simulink model "rfsoc4x2_ospfb_128"  (R2021a)
settings: Solver=VariableStepAuto  StartTime=0.0  StopTime=2048  RelTol=1e-3
undefined symbols (not defined in the file): pfb_coeff_gen_calc
libraries: xbsIndex_r4 x37092, casper_library_delays x737, casper_library_misc x68, xps_library x1
(part 15 of 339)

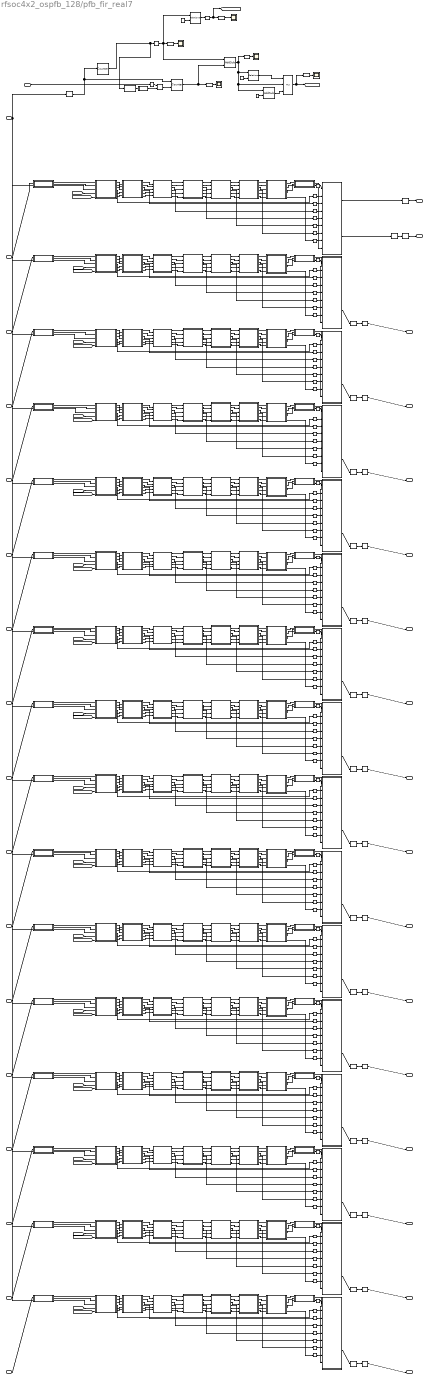
== system rfsoc4x2_ospfb_128/pfb_fir_real7 ==
  note: data 9 first out
  sync : Inport
  pol1_in1 : Inport  Port=2
  pol1_in2 : Inport  Port=3
  pol1_in3 : Inport  Port=4
  pol1_in4 : Inport  Port=5
  pol1_in5 : Inport  Port=6
  pol1_in6 : Inport  Port=7
  pol1_in7 : Inport  Port=8
  pol1_in8 : Inport  Port=9
  pol1_in9 : Inport  Port=10
  pol1_in10 : Inport  Port=11
  pol1_in11 : Inport  Port=12
  pol1_in12 : Inport  Port=13
  pol1_in13 : Inport  Port=14
  pol1_in14 : Inport  Port=15
  pol1_in15 : Inport  Port=16
  pol1_in16 : Inport  Port=17
  en_ctrl : Inport  Port=18
  AddSub11 : xbsIndex_r4/AddSub  mode=Addition  use_carryin=off  use_carryout=off  en=off  latency=0  precision=User Defined  arith_type=Unsigned  n_bits=(log2((2^8 / 2^4)))+1  bin_pt=0  quantization=Truncate  overflow=Wrap  use_behavioral_HDL=off  hw_selection=Fabric  pipelined=off  dbl_ovrd=off  block_type=addsub
  AddSub12 : xbsIndex_r4/AddSub  mode=Subtraction  use_carryin=off  use_carryout=off  en=off  latency=0  precision=User Defined  arith_type=Unsigned  n_bits=log2((2^8 / 2^4))  bin_pt=0  quantization=Truncate  overflow=Wrap  use_behavioral_HDL=off  hw_selection=Fabric  pipelined=off  dbl_ovrd=off  block_type=addsub
  Constant61 : xbsIndex_r4/Constant  const=(2^8 / 2^4) - 1  gui_display_data_type=Fixed-point  arith_type=Unsigned  n_bits=log2((2^8 / 2^4))  bin_pt=0  preci_type=Single  exp_width=8  frac_width=24  explicit_period=off  period=1  equ=P=C  opselect=C  inp2=PCIN>>17  opr=+  inp1=P  carry=CIN  dbl_ovrd=off  block_type=constant
  Constant62 : xbsIndex_r4/Constant  const=(2^8 / 2^4)  gui_display_data_type=Fixed-point  arith_type=Unsigned  n_bits=log2((2^8 / 2^4)) + 1  bin_pt=0  preci_type=Single  exp_width=8  frac_width=24  explicit_period=off  period=1  equ=P=C  opselect=C  inp2=PCIN>>17  opr=+  inp1=P  carry=CIN  dbl_ovrd=off  block_type=constant
  Constant63 : xbsIndex_r4/Constant  const=11  gui_display_data_type=Fixed-point  arith_type=Unsigned  n_bits=4  bin_pt=0  preci_type=Single  exp_width=8  frac_width=24  explicit_period=off  period=1  equ=P=C  opselect=C  inp2=PCIN>>17  opr=+  inp1=P  carry=CIN  dbl_ovrd=off  block_type=constant
  Counter36 : xbsIndex_r4/Counter  cnt_type=Free Running  cnt_to=1023  operation=Down  start_count=0  cnt_by_val=(2^8 / 2^4)/4  arith_type=Unsigned  n_bits=log2((2^8 / 2^4))  bin_pt=0  load_pin=off  rst=on  en=on  explicit_period=on  period=1  use_behavioral_HDL=off  implementation=Fabric  dbl_ovrd=off  block_type=counter
  Counter38 : xbsIndex_r4/Counter  cnt_type=Free Running  cnt_to=1023  operation=Up  start_count=0  cnt_by_val=1  arith_type=Unsigned  n_bits=log2((2^8 / 2^4))  bin_pt=0  load_pin=off  rst=on  en=off  explicit_period=on  period=1  use_behavioral_HDL=off  implementation=Fabric  dbl_ovrd=off  block_type=counter
  Delay26 : xbsIndex_r4/Delay  rst=off  infoeditControl=Selection of Reset will increase slice count due to use of real FFs and instead of SRLs  en=off  latency=1  reg_retiming=off  dbl_ovrd=off  block_type=delay
  Delay27 : xbsIndex_r4/Delay  rst=off  infoeditControl=Selection of Reset will increase slice count due to use of real FFs and instead of SRLs  en=off  latency=4  reg_retiming=off  dbl_ovrd=off  block_type=delay
  Gateway Out{250..253,255} (5 alike) : xbsIndex_r4/Gateway Out  inherit_from_input=off  hdl_port=on  rows=1  columns=1  UseAsDAC=off  DACChannel='1'  interface=None  automatic_assignment=on  address_offset=hex2dec('00')  intf_name=''  intf_description=''  timing_constraint=None  locs_specified=off  LOCs={}  io_standard={}  block_type=gatewayout
  Inverter : xbsIndex_r4/Inverter  en=off  latency=0  dbl_ovrd=off  block_type=inv
  Logical11 : xbsIndex_r4/Logical  logical_function=AND  inputs=2  en=off  latency=0  precision=Full  arith_type=Unsigned  n_bits=16  bin_pt=0  align_bp=on  dbl_ovrd=off  block_type=logical
  Mux3 : xbsIndex_r4/Mux  inputs=2  en=off  latency=0  precision=User Defined  arith_type=Unsigned  n_bits=log2((2^8 / 2^4))  bin_pt=0  quantization=Truncate  overflow=Wrap  dbl_ovrd=off  block_type=mux
  Relational11 : xbsIndex_r4/Relational  mode=a>b  op_type=Bool  en=off  latency=0  dbl_ovrd=off  block_type=relational
  Relational12 : xbsIndex_r4/Relational  mode=a>b  op_type=Bool  en=off  latency=0  dbl_ovrd=off  block_type=relational
  Slice20 : xbsIndex_r4/Slice  nbits=1  boolean_output=on  mode=Upper Bit Location + Width  bit1=0  base1=MSB of Input  bit0=0  base0=LSB of Input  dbl_ovrd=off  block_type=slice
  adder_1_1 : Subsystem  AncestorBlock=casper_library_misc/adder_tree  mask(adder_tree){n_inputs=8, csp_latency=1, adder_imp=Fabric, first_stage_hdl=on, floating_point=off, dvalid_en=off, float_type=single, frac_width=0, exp_width=0}
      mask prompts: n_inputs "Number of Inputs"; csp_latency "Add Latency"; adder_imp "Adder implementation"; first_stage_hdl "Use behavioural HDL for first stage of adders"; floating_point "floating point"; float_type "float type"; frac_width "fraction length"; exp_width "exponent length"
      mask help:
      | Sums all inputs using a tree of adds and delays.
      |
      | Number of inputs: The number of inputs to the block to be summed
      | Add latency: The number of clock cycles to perform one addition (affects timing)..
      | Adder implementation: choice of fabric or DSP48E core, or behavioral HDL
      | Use behavioural HDL for first stage of adders: Causes the first stage of adders to be absorbed into DSP blocks if multipliers precede them (Virtex 5). Overrides Adder implementation
      mask init: same as rfsoc4x2_ospfb_128/pfb_fir_real10/adder_1_1
      settings: AttributesFormatString=latency 3
      mask Help: eval('xlWeb(''http://casper.berkeley.edu/wiki/Adder_tree'')')
      mask TypeOptions adder_imp: Behavioral | Fabric | DSP48
      mask Callback floating_point:
      | onoff = get_param(gcb, 'floating_point');
      | if strcmp(onoff,'on')
      |     enable_fixpt = 'off';
      |     set_param_state(gcb, 'float_type', 'on')
      | 
      |     f_type = get_param(gcb, 'float_type');
      |     if strcmp(f_type,'custom')
      |         set_param_state(gcb, 'exp_width', 'on')
      |         set_param_state(gcb, 'frac_width', 'on')
      |     else
      |         set_param_state(gcb, 'exp_width', 'off')
      |         set_param_state(gcb, 'frac_width', 'off')
      |     end
      | 
      | 
      | else
      |     enable_fixpt = 'on';
      |     set_param_state(gcb, 'float_type', 'off')
      |     set_param_state(gcb, 'exp_width', 'off')
      |     set_param_state(gcb, 'frac_width', 'off')
      | end
      mask TypeOptions float_type: single | custom
      mask Callback float_type:
      | f_type = get_param(gcb, 'float_type');
      | if strcmp(f_type,'custom')
      |     set_param_state(gcb, 'exp_width', 'on')
      |     set_param_state(gcb, 'frac_width', 'on')
      | else
      |     set_param_state(gcb, 'exp_width', 'off')
      |     set_param_state(gcb, 'frac_width', 'off')
      | end
  adder_1_10 : Subsystem  AncestorBlock=casper_library_misc/adder_tree  mask(adder_tree){n_inputs=8, csp_latency=1, adder_imp=Fabric, first_stage_hdl=on, floating_point=off, dvalid_en=off, float_type=single, frac_width=0, exp_width=0}
      mask prompts: n_inputs "Number of Inputs"; csp_latency "Add Latency"; adder_imp "Adder implementation"; first_stage_hdl "Use behavioural HDL for first stage of adders"; floating_point "floating point"; float_type "float type"; frac_width "fraction length"; exp_width "exponent length"
      mask help:
      | Sums all inputs using a tree of adds and delays.
      |
      | Number of inputs: The number of inputs to the block to be summed
      | Add latency: The number of clock cycles to perform one addition (affects timing)..
      | Adder implementation: choice of fabric or DSP48E core, or behavioral HDL
      | Use behavioural HDL for first stage of adders: Causes the first stage of adders to be absorbed into DSP blocks if multipliers precede them (Virtex 5). Overrides Adder implementation
      mask init: same as rfsoc4x2_ospfb_128/pfb_fir_real10/adder_1_1
      settings: AttributesFormatString=latency 3
      mask Help: eval('xlWeb(''http://casper.berkeley.edu/wiki/Adder_tree'')')
      mask TypeOptions adder_imp: Behavioral | Fabric | DSP48
      mask Callback floating_point:
      | onoff = get_param(gcb, 'floating_point');
      | if strcmp(onoff,'on')
      |     enable_fixpt = 'off';
      |     set_param_state(gcb, 'float_type', 'on')
      | 
      |     f_type = get_param(gcb, 'float_type');
      |     if strcmp(f_type,'custom')
      |         set_param_state(gcb, 'exp_width', 'on')
      |         set_param_state(gcb, 'frac_width', 'on')
      |     else
      |         set_param_state(gcb, 'exp_width', 'off')
      |         set_param_state(gcb, 'frac_width', 'off')
      |     end
      | 
      | 
      | else
      |     enable_fixpt = 'on';
      |     set_param_state(gcb, 'float_type', 'off')
      |     set_param_state(gcb, 'exp_width', 'off')
      |     set_param_state(gcb, 'frac_width', 'off')
      | end
      mask TypeOptions float_type: single | custom
      mask Callback float_type:
      | f_type = get_param(gcb, 'float_type');
      | if strcmp(f_type,'custom')
      |     set_param_state(gcb, 'exp_width', 'on')
      |     set_param_state(gcb, 'frac_width', 'on')
      | else
      |     set_param_state(gcb, 'exp_width', 'off')
      |     set_param_state(gcb, 'frac_width', 'off')
      | end
  adder_1_11 : Subsystem  AncestorBlock=casper_library_misc/adder_tree  mask(adder_tree){n_inputs=8, csp_latency=1, adder_imp=Fabric, first_stage_hdl=on, floating_point=off, dvalid_en=off, float_type=single, frac_width=0, exp_width=0}
      mask prompts: n_inputs "Number of Inputs"; csp_latency "Add Latency"; adder_imp "Adder implementation"; first_stage_hdl "Use behavioural HDL for first stage of adders"; floating_point "floating point"; float_type "float type"; frac_width "fraction length"; exp_width "exponent length"
      mask help:
      | Sums all inputs using a tree of adds and delays.
      |
      | Number of inputs: The number of inputs to the block to be summed
      | Add latency: The number of clock cycles to perform one addition (affects timing)..
      | Adder implementation: choice of fabric or DSP48E core, or behavioral HDL
      | Use behavioural HDL for first stage of adders: Causes the first stage of adders to be absorbed into DSP blocks if multipliers precede them (Virtex 5). Overrides Adder implementation
      mask init: same as rfsoc4x2_ospfb_128/pfb_fir_real10/adder_1_1
      settings: AttributesFormatString=latency 3
      mask Help: eval('xlWeb(''http://casper.berkeley.edu/wiki/Adder_tree'')')
      mask TypeOptions adder_imp: Behavioral | Fabric | DSP48
      mask Callback floating_point:
      | onoff = get_param(gcb, 'floating_point');
      | if strcmp(onoff,'on')
      |     enable_fixpt = 'off';
      |     set_param_state(gcb, 'float_type', 'on')
      | 
      |     f_type = get_param(gcb, 'float_type');
      |     if strcmp(f_type,'custom')
      |         set_param_state(gcb, 'exp_width', 'on')
      |         set_param_state(gcb, 'frac_width', 'on')
      |     else
      |         set_param_state(gcb, 'exp_width', 'off')
      |         set_param_state(gcb, 'frac_width', 'off')
      |     end
      | 
      | 
      | else
      |     enable_fixpt = 'on';
      |     set_param_state(gcb, 'float_type', 'off')
      |     set_param_state(gcb, 'exp_width', 'off')
      |     set_param_state(gcb, 'frac_width', 'off')
      | end
      mask TypeOptions float_type: single | custom
      mask Callback float_type:
      | f_type = get_param(gcb, 'float_type');
      | if strcmp(f_type,'custom')
      |     set_param_state(gcb, 'exp_width', 'on')
      |     set_param_state(gcb, 'frac_width', 'on')
      | else
      |     set_param_state(gcb, 'exp_width', 'off')
      |     set_param_state(gcb, 'frac_width', 'off')
      | end
  adder_1_12 : Subsystem  AncestorBlock=casper_library_misc/adder_tree  mask(adder_tree){n_inputs=8, csp_latency=1, adder_imp=Fabric, first_stage_hdl=on, floating_point=off, dvalid_en=off, float_type=single, frac_width=0, exp_width=0}
      mask prompts: n_inputs "Number of Inputs"; csp_latency "Add Latency"; adder_imp "Adder implementation"; first_stage_hdl "Use behavioural HDL for first stage of adders"; floating_point "floating point"; float_type "float type"; frac_width "fraction length"; exp_width "exponent length"
      mask help:
      | Sums all inputs using a tree of adds and delays.
      |
      | Number of inputs: The number of inputs to the block to be summed
      | Add latency: The number of clock cycles to perform one addition (affects timing)..
      | Adder implementation: choice of fabric or DSP48E core, or behavioral HDL
      | Use behavioural HDL for first stage of adders: Causes the first stage of adders to be absorbed into DSP blocks if multipliers precede them (Virtex 5). Overrides Adder implementation
      mask init: same as rfsoc4x2_ospfb_128/pfb_fir_real10/adder_1_1
      settings: AttributesFormatString=latency 3
      mask Help: eval('xlWeb(''http://casper.berkeley.edu/wiki/Adder_tree'')')
      mask TypeOptions adder_imp: Behavioral | Fabric | DSP48
      mask Callback floating_point:
      | onoff = get_param(gcb, 'floating_point');
      | if strcmp(onoff,'on')
      |     enable_fixpt = 'off';
      |     set_param_state(gcb, 'float_type', 'on')
      | 
      |     f_type = get_param(gcb, 'float_type');
      |     if strcmp(f_type,'custom')
      |         set_param_state(gcb, 'exp_width', 'on')
      |         set_param_state(gcb, 'frac_width', 'on')
      |     else
      |         set_param_state(gcb, 'exp_width', 'off')
      |         set_param_state(gcb, 'frac_width', 'off')
      |     end
      | 
      | 
      | else
      |     enable_fixpt = 'on';
      |     set_param_state(gcb, 'float_type', 'off')
      |     set_param_state(gcb, 'exp_width', 'off')
      |     set_param_state(gcb, 'frac_width', 'off')
      | end
      mask TypeOptions float_type: single | custom
      mask Callback float_type:
      | f_type = get_param(gcb, 'float_type');
      | if strcmp(f_type,'custom')
      |     set_param_state(gcb, 'exp_width', 'on')
      |     set_param_state(gcb, 'frac_width', 'on')
      | else
      |     set_param_state(gcb, 'exp_width', 'off')
      |     set_param_state(gcb, 'frac_width', 'off')
      | end
  adder_1_13 : Subsystem  AncestorBlock=casper_library_misc/adder_tree  mask(adder_tree){n_inputs=8, csp_latency=1, adder_imp=Fabric, first_stage_hdl=on, floating_point=off, dvalid_en=off, float_type=single, frac_width=0, exp_width=0}
      mask prompts: n_inputs "Number of Inputs"; csp_latency "Add Latency"; adder_imp "Adder implementation"; first_stage_hdl "Use behavioural HDL for first stage of adders"; floating_point "floating point"; float_type "float type"; frac_width "fraction length"; exp_width "exponent length"
      mask help:
      | Sums all inputs using a tree of adds and delays.
      |
      | Number of inputs: The number of inputs to the block to be summed
      | Add latency: The number of clock cycles to perform one addition (affects timing)..
      | Adder implementation: choice of fabric or DSP48E core, or behavioral HDL
      | Use behavioural HDL for first stage of adders: Causes the first stage of adders to be absorbed into DSP blocks if multipliers precede them (Virtex 5). Overrides Adder implementation
      mask init: same as rfsoc4x2_ospfb_128/pfb_fir_real10/adder_1_1
      settings: AttributesFormatString=latency 3
      mask Help: eval('xlWeb(''http://casper.berkeley.edu/wiki/Adder_tree'')')
      mask TypeOptions adder_imp: Behavioral | Fabric | DSP48
      mask Callback floating_point:
      | onoff = get_param(gcb, 'floating_point');
      | if strcmp(onoff,'on')
      |     enable_fixpt = 'off';
      |     set_param_state(gcb, 'float_type', 'on')
      | 
      |     f_type = get_param(gcb, 'float_type');
      |     if strcmp(f_type,'custom')
      |         set_param_state(gcb, 'exp_width', 'on')
      |         set_param_state(gcb, 'frac_width', 'on')
      |     else
      |         set_param_state(gcb, 'exp_width', 'off')
      |         set_param_state(gcb, 'frac_width', 'off')
      |     end
      | 
      | 
      | else
      |     enable_fixpt = 'on';
      |     set_param_state(gcb, 'float_type', 'off')
      |     set_param_state(gcb, 'exp_width', 'off')
      |     set_param_state(gcb, 'frac_width', 'off')
      | end
      mask TypeOptions float_type: single | custom
      mask Callback float_type:
      | f_type = get_param(gcb, 'float_type');
      | if strcmp(f_type,'custom')
      |     set_param_state(gcb, 'exp_width', 'on')
      |     set_param_state(gcb, 'frac_width', 'on')
      | else
      |     set_param_state(gcb, 'exp_width', 'off')
      |     set_param_state(gcb, 'frac_width', 'off')
      | end
  adder_1_14 : Subsystem  AncestorBlock=casper_library_misc/adder_tree  mask(adder_tree){n_inputs=8, csp_latency=1, adder_imp=Fabric, first_stage_hdl=on, floating_point=off, dvalid_en=off, float_type=single, frac_width=0, exp_width=0}
      mask prompts: n_inputs "Number of Inputs"; csp_latency "Add Latency"; adder_imp "Adder implementation"; first_stage_hdl "Use behavioural HDL for first stage of adders"; floating_point "floating point"; float_type "float type"; frac_width "fraction length"; exp_width "exponent length"
      mask help:
      | Sums all inputs using a tree of adds and delays.
      |
      | Number of inputs: The number of inputs to the block to be summed
      | Add latency: The number of clock cycles to perform one addition (affects timing)..
      | Adder implementation: choice of fabric or DSP48E core, or behavioral HDL
      | Use behavioural HDL for first stage of adders: Causes the first stage of adders to be absorbed into DSP blocks if multipliers precede them (Virtex 5). Overrides Adder implementation
      mask init: same as rfsoc4x2_ospfb_128/pfb_fir_real10/adder_1_1
      settings: AttributesFormatString=latency 3
      mask Help: eval('xlWeb(''http://casper.berkeley.edu/wiki/Adder_tree'')')
      mask TypeOptions adder_imp: Behavioral | Fabric | DSP48
      mask Callback floating_point:
      | onoff = get_param(gcb, 'floating_point');
      | if strcmp(onoff,'on')
      |     enable_fixpt = 'off';
      |     set_param_state(gcb, 'float_type', 'on')
      | 
      |     f_type = get_param(gcb, 'float_type');
      |     if strcmp(f_type,'custom')
      |         set_param_state(gcb, 'exp_width', 'on')
      |         set_param_state(gcb, 'frac_width', 'on')
      |     else
      |         set_param_state(gcb, 'exp_width', 'off')
      |         set_param_state(gcb, 'frac_width', 'off')
      |     end
      | 
      | 
      | else
      |     enable_fixpt = 'on';
      |     set_param_state(gcb, 'float_type', 'off')
      |     set_param_state(gcb, 'exp_width', 'off')
      |     set_param_state(gcb, 'frac_width', 'off')
      | end
      mask TypeOptions float_type: single | custom
      mask Callback float_type:
      | f_type = get_param(gcb, 'float_type');
      | if strcmp(f_type,'custom')
      |     set_param_state(gcb, 'exp_width', 'on')
      |     set_param_state(gcb, 'frac_width', 'on')
      | else
      |     set_param_state(gcb, 'exp_width', 'off')
      |     set_param_state(gcb, 'frac_width', 'off')
      | end
  adder_1_15 : Subsystem  AncestorBlock=casper_library_misc/adder_tree  mask(adder_tree){n_inputs=8, csp_latency=1, adder_imp=Fabric, first_stage_hdl=on, floating_point=off, dvalid_en=off, float_type=single, frac_width=0, exp_width=0}
      mask prompts: n_inputs "Number of Inputs"; csp_latency "Add Latency"; adder_imp "Adder implementation"; first_stage_hdl "Use behavioural HDL for first stage of adders"; floating_point "floating point"; float_type "float type"; frac_width "fraction length"; exp_width "exponent length"
      mask help:
      | Sums all inputs using a tree of adds and delays.
      |
      | Number of inputs: The number of inputs to the block to be summed
      | Add latency: The number of clock cycles to perform one addition (affects timing)..
      | Adder implementation: choice of fabric or DSP48E core, or behavioral HDL
      | Use behavioural HDL for first stage of adders: Causes the first stage of adders to be absorbed into DSP blocks if multipliers precede them (Virtex 5). Overrides Adder implementation
      mask init: same as rfsoc4x2_ospfb_128/pfb_fir_real10/adder_1_1
      settings: AttributesFormatString=latency 3
      mask Help: eval('xlWeb(''http://casper.berkeley.edu/wiki/Adder_tree'')')
      mask TypeOptions adder_imp: Behavioral | Fabric | DSP48
      mask Callback floating_point:
      | onoff = get_param(gcb, 'floating_point');
      | if strcmp(onoff,'on')
      |     enable_fixpt = 'off';
      |     set_param_state(gcb, 'float_type', 'on')
      | 
      |     f_type = get_param(gcb, 'float_type');
      |     if strcmp(f_type,'custom')
      |         set_param_state(gcb, 'exp_width', 'on')
      |         set_param_state(gcb, 'frac_width', 'on')
      |     else
      |         set_param_state(gcb, 'exp_width', 'off')
      |         set_param_state(gcb, 'frac_width', 'off')
      |     end
      | 
      | 
      | else
      |     enable_fixpt = 'on';
      |     set_param_state(gcb, 'float_type', 'off')
      |     set_param_state(gcb, 'exp_width', 'off')
      |     set_param_state(gcb, 'frac_width', 'off')
      | end
      mask TypeOptions float_type: single | custom
      mask Callback float_type:
      | f_type = get_param(gcb, 'float_type');
      | if strcmp(f_type,'custom')
      |     set_param_state(gcb, 'exp_width', 'on')
      |     set_param_state(gcb, 'frac_width', 'on')
      | else
      |     set_param_state(gcb, 'exp_width', 'off')
      |     set_param_state(gcb, 'frac_width', 'off')
      | end
  adder_1_16 : Subsystem  AncestorBlock=casper_library_misc/adder_tree  mask(adder_tree){n_inputs=8, csp_latency=1, adder_imp=Fabric, first_stage_hdl=on, floating_point=off, dvalid_en=off, float_type=single, frac_width=0, exp_width=0}
      mask prompts: n_inputs "Number of Inputs"; csp_latency "Add Latency"; adder_imp "Adder implementation"; first_stage_hdl "Use behavioural HDL for first stage of adders"; floating_point "floating point"; float_type "float type"; frac_width "fraction length"; exp_width "exponent length"
      mask help:
      | Sums all inputs using a tree of adds and delays.
      |
      | Number of inputs: The number of inputs to the block to be summed
      | Add latency: The number of clock cycles to perform one addition (affects timing)..
      | Adder implementation: choice of fabric or DSP48E core, or behavioral HDL
      | Use behavioural HDL for first stage of adders: Causes the first stage of adders to be absorbed into DSP blocks if multipliers precede them (Virtex 5). Overrides Adder implementation
      mask init: same as rfsoc4x2_ospfb_128/pfb_fir_real10/adder_1_1
      settings: AttributesFormatString=latency 3
      mask Help: eval('xlWeb(''http://casper.berkeley.edu/wiki/Adder_tree'')')
      mask TypeOptions adder_imp: Behavioral | Fabric | DSP48
      mask Callback floating_point:
      | onoff = get_param(gcb, 'floating_point');
      | if strcmp(onoff,'on')
      |     enable_fixpt = 'off';
      |     set_param_state(gcb, 'float_type', 'on')
      | 
      |     f_type = get_param(gcb, 'float_type');
      |     if strcmp(f_type,'custom')
      |         set_param_state(gcb, 'exp_width', 'on')
      |         set_param_state(gcb, 'frac_width', 'on')
      |     else
      |         set_param_state(gcb, 'exp_width', 'off')
      |         set_param_state(gcb, 'frac_width', 'off')
      |     end
      | 
      | 
      | else
      |     enable_fixpt = 'on';
      |     set_param_state(gcb, 'float_type', 'off')
      |     set_param_state(gcb, 'exp_width', 'off')
      |     set_param_state(gcb, 'frac_width', 'off')
      | end
      mask TypeOptions float_type: single | custom
      mask Callback float_type:
      | f_type = get_param(gcb, 'float_type');
      | if strcmp(f_type,'custom')
      |     set_param_state(gcb, 'exp_width', 'on')
      |     set_param_state(gcb, 'frac_width', 'on')
      | else
      |     set_param_state(gcb, 'exp_width', 'off')
      |     set_param_state(gcb, 'frac_width', 'off')
      | end
  adder_1_2 : Subsystem  AncestorBlock=casper_library_misc/adder_tree  mask(adder_tree){n_inputs=8, csp_latency=1, adder_imp=Fabric, first_stage_hdl=on, floating_point=off, dvalid_en=off, float_type=single, frac_width=0, exp_width=0}
      mask prompts: n_inputs "Number of Inputs"; csp_latency "Add Latency"; adder_imp "Adder implementation"; first_stage_hdl "Use behavioural HDL for first stage of adders"; floating_point "floating point"; float_type "float type"; frac_width "fraction length"; exp_width "exponent length"
      mask help:
      | Sums all inputs using a tree of adds and delays.
      |
      | Number of inputs: The number of inputs to the block to be summed
      | Add latency: The number of clock cycles to perform one addition (affects timing)..
      | Adder implementation: choice of fabric or DSP48E core, or behavioral HDL
      | Use behavioural HDL for first stage of adders: Causes the first stage of adders to be absorbed into DSP blocks if multipliers precede them (Virtex 5). Overrides Adder implementation
      mask init: same as rfsoc4x2_ospfb_128/pfb_fir_real10/adder_1_1
      settings: AttributesFormatString=latency 3
      mask Help: eval('xlWeb(''http://casper.berkeley.edu/wiki/Adder_tree'')')
      mask TypeOptions adder_imp: Behavioral | Fabric | DSP48
      mask Callback floating_point:
      | onoff = get_param(gcb, 'floating_point');
      | if strcmp(onoff,'on')
      |     enable_fixpt = 'off';
      |     set_param_state(gcb, 'float_type', 'on')
      | 
      |     f_type = get_param(gcb, 'float_type');
      |     if strcmp(f_type,'custom')
      |         set_param_state(gcb, 'exp_width', 'on')
      |         set_param_state(gcb, 'frac_width', 'on')
      |     else
      |         set_param_state(gcb, 'exp_width', 'off')
      |         set_param_state(gcb, 'frac_width', 'off')
      |     end
      | 
      | 
      | else
      |     enable_fixpt = 'on';
      |     set_param_state(gcb, 'float_type', 'off')
      |     set_param_state(gcb, 'exp_width', 'off')
      |     set_param_state(gcb, 'frac_width', 'off')
      | end
      mask TypeOptions float_type: single | custom
      mask Callback float_type:
      | f_type = get_param(gcb, 'float_type');
      | if strcmp(f_type,'custom')
      |     set_param_state(gcb, 'exp_width', 'on')
      |     set_param_state(gcb, 'frac_width', 'on')
      | else
      |     set_param_state(gcb, 'exp_width', 'off')
      |     set_param_state(gcb, 'frac_width', 'off')
      | end
  adder_1_3 : Subsystem  AncestorBlock=casper_library_misc/adder_tree  mask(adder_tree){n_inputs=8, csp_latency=1, adder_imp=Fabric, first_stage_hdl=on, floating_point=off, dvalid_en=off, float_type=single, frac_width=0, exp_width=0}
      mask prompts: n_inputs "Number of Inputs"; csp_latency "Add Latency"; adder_imp "Adder implementation"; first_stage_hdl "Use behavioural HDL for first stage of adders"; floating_point "floating point"; float_type "float type"; frac_width "fraction length"; exp_width "exponent length"
      mask help:
      | Sums all inputs using a tree of adds and delays.
      |
      | Number of inputs: The number of inputs to the block to be summed
      | Add latency: The number of clock cycles to perform one addition (affects timing)..
      | Adder implementation: choice of fabric or DSP48E core, or behavioral HDL
      | Use behavioural HDL for first stage of adders: Causes the first stage of adders to be absorbed into DSP blocks if multipliers precede them (Virtex 5). Overrides Adder implementation
      mask init: same as rfsoc4x2_ospfb_128/pfb_fir_real10/adder_1_1
      settings: AttributesFormatString=latency 3
      mask Help: eval('xlWeb(''http://casper.berkeley.edu/wiki/Adder_tree'')')
      mask TypeOptions adder_imp: Behavioral | Fabric | DSP48
      mask Callback floating_point:
      | onoff = get_param(gcb, 'floating_point');
      | if strcmp(onoff,'on')
      |     enable_fixpt = 'off';
      |     set_param_state(gcb, 'float_type', 'on')
      | 
      |     f_type = get_param(gcb, 'float_type');
      |     if strcmp(f_type,'custom')
      |         set_param_state(gcb, 'exp_width', 'on')
      |         set_param_state(gcb, 'frac_width', 'on')
      |     else
      |         set_param_state(gcb, 'exp_width', 'off')
      |         set_param_state(gcb, 'frac_width', 'off')
      |     end
      | 
      | 
      | else
      |     enable_fixpt = 'on';
      |     set_param_state(gcb, 'float_type', 'off')
      |     set_param_state(gcb, 'exp_width', 'off')
      |     set_param_state(gcb, 'frac_width', 'off')
      | end
      mask TypeOptions float_type: single | custom
      mask Callback float_type:
      | f_type = get_param(gcb, 'float_type');
      | if strcmp(f_type,'custom')
      |     set_param_state(gcb, 'exp_width', 'on')
      |     set_param_state(gcb, 'frac_width', 'on')
      | else
      |     set_param_state(gcb, 'exp_width', 'off')
      |     set_param_state(gcb, 'frac_width', 'off')
      | end
  adder_1_4 : Subsystem  AncestorBlock=casper_library_misc/adder_tree  mask(adder_tree){n_inputs=8, csp_latency=1, adder_imp=Fabric, first_stage_hdl=on, floating_point=off, dvalid_en=off, float_type=single, frac_width=0, exp_width=0}
      mask prompts: n_inputs "Number of Inputs"; csp_latency "Add Latency"; adder_imp "Adder implementation"; first_stage_hdl "Use behavioural HDL for first stage of adders"; floating_point "floating point"; float_type "float type"; frac_width "fraction length"; exp_width "exponent length"
      mask help:
      | Sums all inputs using a tree of adds and delays.
      |
      | Number of inputs: The number of inputs to the block to be summed
      | Add latency: The number of clock cycles to perform one addition (affects timing)..
      | Adder implementation: choice of fabric or DSP48E core, or behavioral HDL
      | Use behavioural HDL for first stage of adders: Causes the first stage of adders to be absorbed into DSP blocks if multipliers precede them (Virtex 5). Overrides Adder implementation
      mask init: same as rfsoc4x2_ospfb_128/pfb_fir_real10/adder_1_1
      settings: AttributesFormatString=latency 3
      mask Help: eval('xlWeb(''http://casper.berkeley.edu/wiki/Adder_tree'')')
      mask TypeOptions adder_imp: Behavioral | Fabric | DSP48
      mask Callback floating_point:
      | onoff = get_param(gcb, 'floating_point');
      | if strcmp(onoff,'on')
      |     enable_fixpt = 'off';
      |     set_param_state(gcb, 'float_type', 'on')
      | 
      |     f_type = get_param(gcb, 'float_type');
      |     if strcmp(f_type,'custom')
      |         set_param_state(gcb, 'exp_width', 'on')
      |         set_param_state(gcb, 'frac_width', 'on')
      |     else
      |         set_param_state(gcb, 'exp_width', 'off')
      |         set_param_state(gcb, 'frac_width', 'off')
      |     end
      | 
      | 
      | else
      |     enable_fixpt = 'on';
      |     set_param_state(gcb, 'float_type', 'off')
      |     set_param_state(gcb, 'exp_width', 'off')
      |     set_param_state(gcb, 'frac_width', 'off')
      | end
      mask TypeOptions float_type: single | custom
      mask Callback float_type:
      | f_type = get_param(gcb, 'float_type');
      | if strcmp(f_type,'custom')
      |     set_param_state(gcb, 'exp_width', 'on')
      |     set_param_state(gcb, 'frac_width', 'on')
      | else
      |     set_param_state(gcb, 'exp_width', 'off')
      |     set_param_state(gcb, 'frac_width', 'off')
      | end
  adder_1_5 : Subsystem  AncestorBlock=casper_library_misc/adder_tree  mask(adder_tree){n_inputs=8, csp_latency=1, adder_imp=Fabric, first_stage_hdl=on, floating_point=off, dvalid_en=off, float_type=single, frac_width=0, exp_width=0}
      mask prompts: n_inputs "Number of Inputs"; csp_latency "Add Latency"; adder_imp "Adder implementation"; first_stage_hdl "Use behavioural HDL for first stage of adders"; floating_point "floating point"; float_type "float type"; frac_width "fraction length"; exp_width "exponent length"
      mask help:
      | Sums all inputs using a tree of adds and delays.
      |
      | Number of inputs: The number of inputs to the block to be summed
      | Add latency: The number of clock cycles to perform one addition (affects timing)..
      | Adder implementation: choice of fabric or DSP48E core, or behavioral HDL
      | Use behavioural HDL for first stage of adders: Causes the first stage of adders to be absorbed into DSP blocks if multipliers precede them (Virtex 5). Overrides Adder implementation
      mask init: same as rfsoc4x2_ospfb_128/pfb_fir_real10/adder_1_1
      settings: AttributesFormatString=latency 3
      mask Help: eval('xlWeb(''http://casper.berkeley.edu/wiki/Adder_tree'')')
      mask TypeOptions adder_imp: Behavioral | Fabric | DSP48
      mask Callback floating_point:
      | onoff = get_param(gcb, 'floating_point');
      | if strcmp(onoff,'on')
      |     enable_fixpt = 'off';
      |     set_param_state(gcb, 'float_type', 'on')
      | 
      |     f_type = get_param(gcb, 'float_type');
      |     if strcmp(f_type,'custom')
      |         set_param_state(gcb, 'exp_width', 'on')
      |         set_param_state(gcb, 'frac_width', 'on')
      |     else
      |         set_param_state(gcb, 'exp_width', 'off')
      |         set_param_state(gcb, 'frac_width', 'off')
      |     end
      | 
      | 
      | else
      |     enable_fixpt = 'on';
      |     set_param_state(gcb, 'float_type', 'off')
      |     set_param_state(gcb, 'exp_width', 'off')
      |     set_param_state(gcb, 'frac_width', 'off')
      | end
      mask TypeOptions float_type: single | custom
      mask Callback float_type:
      | f_type = get_param(gcb, 'float_type');
      | if strcmp(f_type,'custom')
      |     set_param_state(gcb, 'exp_width', 'on')
      |     set_param_state(gcb, 'frac_width', 'on')
      | else
      |     set_param_state(gcb, 'exp_width', 'off')
      |     set_param_state(gcb, 'frac_width', 'off')
      | end
  adder_1_6 : Subsystem  AncestorBlock=casper_library_misc/adder_tree  mask(adder_tree){n_inputs=8, csp_latency=1, adder_imp=Fabric, first_stage_hdl=on, floating_point=off, dvalid_en=off, float_type=single, frac_width=0, exp_width=0}
      mask prompts: n_inputs "Number of Inputs"; csp_latency "Add Latency"; adder_imp "Adder implementation"; first_stage_hdl "Use behavioural HDL for first stage of adders"; floating_point "floating point"; float_type "float type"; frac_width "fraction length"; exp_width "exponent length"
      mask help:
      | Sums all inputs using a tree of adds and delays.
      |
      | Number of inputs: The number of inputs to the block to be summed
      | Add latency: The number of clock cycles to perform one addition (affects timing)..
      | Adder implementation: choice of fabric or DSP48E core, or behavioral HDL
      | Use behavioural HDL for first stage of adders: Causes the first stage of adders to be absorbed into DSP blocks if multipliers precede them (Virtex 5). Overrides Adder implementation
      mask init: same as rfsoc4x2_ospfb_128/pfb_fir_real10/adder_1_1
      settings: AttributesFormatString=latency 3
      mask Help: eval('xlWeb(''http://casper.berkeley.edu/wiki/Adder_tree'')')
      mask TypeOptions adder_imp: Behavioral | Fabric | DSP48
      mask Callback floating_point:
      | onoff = get_param(gcb, 'floating_point');
      | if strcmp(onoff,'on')
      |     enable_fixpt = 'off';
      |     set_param_state(gcb, 'float_type', 'on')
      | 
      |     f_type = get_param(gcb, 'float_type');
      |     if strcmp(f_type,'custom')
      |         set_param_state(gcb, 'exp_width', 'on')
      |         set_param_state(gcb, 'frac_width', 'on')
      |     else
      |         set_param_state(gcb, 'exp_width', 'off')
      |         set_param_state(gcb, 'frac_width', 'off')
      |     end
      | 
      | 
      | else
      |     enable_fixpt = 'on';
      |     set_param_state(gcb, 'float_type', 'off')
      |     set_param_state(gcb, 'exp_width', 'off')
      |     set_param_state(gcb, 'frac_width', 'off')
      | end
      mask TypeOptions float_type: single | custom
      mask Callback float_type:
      | f_type = get_param(gcb, 'float_type');
      | if strcmp(f_type,'custom')
      |     set_param_state(gcb, 'exp_width', 'on')
      |     set_param_state(gcb, 'frac_width', 'on')
      | else
      |     set_param_state(gcb, 'exp_width', 'off')
      |     set_param_state(gcb, 'frac_width', 'off')
      | end
  adder_1_7 : Subsystem  AncestorBlock=casper_library_misc/adder_tree  mask(adder_tree){n_inputs=8, csp_latency=1, adder_imp=Fabric, first_stage_hdl=on, floating_point=off, dvalid_en=off, float_type=single, frac_width=0, exp_width=0}
      mask prompts: n_inputs "Number of Inputs"; csp_latency "Add Latency"; adder_imp "Adder implementation"; first_stage_hdl "Use behavioural HDL for first stage of adders"; floating_point "floating point"; float_type "float type"; frac_width "fraction length"; exp_width "exponent length"
      mask help:
      | Sums all inputs using a tree of adds and delays.
      |
      | Number of inputs: The number of inputs to the block to be summed
      | Add latency: The number of clock cycles to perform one addition (affects timing)..
      | Adder implementation: choice of fabric or DSP48E core, or behavioral HDL
      | Use behavioural HDL for first stage of adders: Causes the first stage of adders to be absorbed into DSP blocks if multipliers precede them (Virtex 5). Overrides Adder implementation
      mask init: same as rfsoc4x2_ospfb_128/pfb_fir_real10/adder_1_1
      settings: AttributesFormatString=latency 3
      mask Help: eval('xlWeb(''http://casper.berkeley.edu/wiki/Adder_tree'')')
      mask TypeOptions adder_imp: Behavioral | Fabric | DSP48
      mask Callback floating_point:
      | onoff = get_param(gcb, 'floating_point');
      | if strcmp(onoff,'on')
      |     enable_fixpt = 'off';
      |     set_param_state(gcb, 'float_type', 'on')
      | 
      |     f_type = get_param(gcb, 'float_type');
      |     if strcmp(f_type,'custom')
      |         set_param_state(gcb, 'exp_width', 'on')
      |         set_param_state(gcb, 'frac_width', 'on')
      |     else
      |         set_param_state(gcb, 'exp_width', 'off')
      |         set_param_state(gcb, 'frac_width', 'off')
      |     end
      | 
      | 
      | else
      |     enable_fixpt = 'on';
      |     set_param_state(gcb, 'float_type', 'off')
      |     set_param_state(gcb, 'exp_width', 'off')
      |     set_param_state(gcb, 'frac_width', 'off')
      | end
      mask TypeOptions float_type: single | custom
      mask Callback float_type:
      | f_type = get_param(gcb, 'float_type');
      | if strcmp(f_type,'custom')
      |     set_param_state(gcb, 'exp_width', 'on')
      |     set_param_state(gcb, 'frac_width', 'on')
      | else
      |     set_param_state(gcb, 'exp_width', 'off')
      |     set_param_state(gcb, 'frac_width', 'off')
      | end
  adder_1_8 : Subsystem  AncestorBlock=casper_library_misc/adder_tree  mask(adder_tree){n_inputs=8, csp_latency=1, adder_imp=Fabric, first_stage_hdl=on, floating_point=off, dvalid_en=off, float_type=single, frac_width=0, exp_width=0}
      mask prompts: n_inputs "Number of Inputs"; csp_latency "Add Latency"; adder_imp "Adder implementation"; first_stage_hdl "Use behavioural HDL for first stage of adders"; floating_point "floating point"; float_type "float type"; frac_width "fraction length"; exp_width "exponent length"
      mask help:
      | Sums all inputs using a tree of adds and delays.
      |
      | Number of inputs: The number of inputs to the block to be summed
      | Add latency: The number of clock cycles to perform one addition (affects timing)..
      | Adder implementation: choice of fabric or DSP48E core, or behavioral HDL
      | Use behavioural HDL for first stage of adders: Causes the first stage of adders to be absorbed into DSP blocks if multipliers precede them (Virtex 5). Overrides Adder implementation
      mask init: same as rfsoc4x2_ospfb_128/pfb_fir_real10/adder_1_1
      settings: AttributesFormatString=latency 3
      mask Help: eval('xlWeb(''http://casper.berkeley.edu/wiki/Adder_tree'')')
      mask TypeOptions adder_imp: Behavioral | Fabric | DSP48
      mask Callback floating_point:
      | onoff = get_param(gcb, 'floating_point');
      | if strcmp(onoff,'on')
      |     enable_fixpt = 'off';
      |     set_param_state(gcb, 'float_type', 'on')
      | 
      |     f_type = get_param(gcb, 'float_type');
      |     if strcmp(f_type,'custom')
      |         set_param_state(gcb, 'exp_width', 'on')
      |         set_param_state(gcb, 'frac_width', 'on')
      |     else
      |         set_param_state(gcb, 'exp_width', 'off')
      |         set_param_state(gcb, 'frac_width', 'off')
      |     end
      | 
      | 
      | else
      |     enable_fixpt = 'on';
      |     set_param_state(gcb, 'float_type', 'off')
      |     set_param_state(gcb, 'exp_width', 'off')
      |     set_param_state(gcb, 'frac_width', 'off')
      | end
      mask TypeOptions float_type: single | custom
      mask Callback float_type:
      | f_type = get_param(gcb, 'float_type');
      | if strcmp(f_type,'custom')
      |     set_param_state(gcb, 'exp_width', 'on')
      |     set_param_state(gcb, 'frac_width', 'on')
      | else
      |     set_param_state(gcb, 'exp_width', 'off')
      |     set_param_state(gcb, 'frac_width', 'off')
      | end
  adder_1_9 : Subsystem  AncestorBlock=casper_library_misc/adder_tree  mask(adder_tree){n_inputs=8, csp_latency=1, adder_imp=Fabric, first_stage_hdl=on, floating_point=off, dvalid_en=off, float_type=single, frac_width=0, exp_width=0}
      mask prompts: n_inputs "Number of Inputs"; csp_latency "Add Latency"; adder_imp "Adder implementation"; first_stage_hdl "Use behavioural HDL for first stage of adders"; floating_point "floating point"; float_type "float type"; frac_width "fraction length"; exp_width "exponent length"
      mask help:
      | Sums all inputs using a tree of adds and delays.
      |
      | Number of inputs: The number of inputs to the block to be summed
      | Add latency: The number of clock cycles to perform one addition (affects timing)..
      | Adder implementation: choice of fabric or DSP48E core, or behavioral HDL
      | Use behavioural HDL for first stage of adders: Causes the first stage of adders to be absorbed into DSP blocks if multipliers precede them (Virtex 5). Overrides Adder implementation
      mask init: same as rfsoc4x2_ospfb_128/pfb_fir_real10/adder_1_1
      settings: AttributesFormatString=latency 3
      mask Help: eval('xlWeb(''http://casper.berkeley.edu/wiki/Adder_tree'')')
      mask TypeOptions adder_imp: Behavioral | Fabric | DSP48
      mask Callback floating_point:
      | onoff = get_param(gcb, 'floating_point');
      | if strcmp(onoff,'on')
      |     enable_fixpt = 'off';
      |     set_param_state(gcb, 'float_type', 'on')
      | 
      |     f_type = get_param(gcb, 'float_type');
      |     if strcmp(f_type,'custom')
      |         set_param_state(gcb, 'exp_width', 'on')
      |         set_param_state(gcb, 'frac_width', 'on')
      |     else
      |         set_param_state(gcb, 'exp_width', 'off')
      |         set_param_state(gcb, 'frac_width', 'off')
      |     end
      | 
      | 
      | else
      |     enable_fixpt = 'on';
      |     set_param_state(gcb, 'float_type', 'off')
      |     set_param_state(gcb, 'exp_width', 'off')
      |     set_param_state(gcb, 'frac_width', 'off')
      | end
      mask TypeOptions float_type: single | custom
      mask Callback float_type:
      | f_type = get_param(gcb, 'float_type');
      | if strcmp(f_type,'custom')
      |     set_param_state(gcb, 'exp_width', 'on')
      |     set_param_state(gcb, 'frac_width', 'on')
      | else
      |     set_param_state(gcb, 'exp_width', 'off')
      |     set_param_state(gcb, 'frac_width', 'off')
      | end
  convert_1_{1..16} (16 alike) : xbsIndex_r4/Convert  gui_display_data_type=Fixed-point  arith_type="Signed  (2's comp)"  n_bits=18  bin_pt=17  float_type=Single  exp_bits=8  fraction_bits=24  quantization="Round  (unbiased: Even Values)"  overflow=Wrap  en=off  latency=1  pipeline=on  dbl_ovrd=off  block_type=convert
  delay{1,3,12,18,28,36,44,52,60,68,76,84,92,100,108,116,124} (17 alike) : xbsIndex_r4/Delay  rst=off  infoeditControl=Selection of Reset will increase slice count due to use of real FFs and instead of SRLs  en=off  latency=1  reg_retiming=off  dbl_ovrd=off  block_type=delay
  delay{9..11,24..27,34..35,42..43,50..51,58..59,66..67,74..75,82..83,90..91,98..99,106..107,114..115,122..123,130} (32 alike) : xbsIndex_r4/Delay  rst=off  infoeditControl=Selection of Reset will increase slice count due to use of real FFs and instead of SRLs  en=off  latency=7  reg_retiming=off  dbl_ovrd=off  block_type=delay
  delay{4,13,19,29,37,45,53,61,69,77,85,93,101,109,117,125} (16 alike) : xbsIndex_r4/Delay  rst=off  infoeditControl=Selection of Reset will increase slice count due to use of real FFs and instead of SRLs  en=off  latency=2  reg_retiming=off  dbl_ovrd=off  block_type=delay
  delay{2,5,14,20,30,38,46,54,62,70,78,86,94,102,110,118,126} (17 alike) : xbsIndex_r4/Delay  rst=off  infoeditControl=Selection of Reset will increase slice count due to use of real FFs and instead of SRLs  en=off  latency=3  reg_retiming=off  dbl_ovrd=off  block_type=delay
  delay{6,15,21,31,39,47,55,63,71,79,87,95,103,111,119,127} (16 alike) : xbsIndex_r4/Delay  rst=off  infoeditControl=Selection of Reset will increase slice count due to use of real FFs and instead of SRLs  en=off  latency=4  reg_retiming=off  dbl_ovrd=off  block_type=delay
  delay{7,16,22,32,40,48,56,64,72,80,88,96,104,112,120,128} (16 alike) : xbsIndex_r4/Delay  rst=off  infoeditControl=Selection of Reset will increase slice count due to use of real FFs and instead of SRLs  en=off  latency=5  reg_retiming=off  dbl_ovrd=off  block_type=delay
  delay{8,17,23,33,41,49,57,65,73,81,89,97,105,113,121,129} (16 alike) : xbsIndex_r4/Delay  rst=off  infoeditControl=Selection of Reset will increase slice count due to use of real FFs and instead of SRLs  en=off  latency=6  reg_retiming=off  dbl_ovrd=off  block_type=delay
  edge_detect8 : Subsystem  AncestorBlock=casper_library_misc/edge_detect  mask(edge_detect){edge=Falling, polarity=Active High, x_in=[0 0.08 0.08 0.16 0.16 0.24 0.24 0.32 0.32 0.4], y_in=[-1 -1  1  1  1  1  1  1  1  1], x_out=[0.6 0.68 0.68 0.76 0.76 0.84 0.84 0.92 0.92 1], y_out=[-1 -1  1  1 -1 -1 -1 -1 -1 -1]}
      mask prompts: edge "Edge Type"; polarity "Output Polarity"; x_in "Input X Positions"; y_in "Input Y Positions"; x_out "Output X Positions"; y_out "Output Y Positions"
      mask help: Output is active for one-cycle after each edge of the specified type (i.e. rising, falling or both).
      mask init: same as rfsoc4x2_ospfb_128/edge_detect10
      settings: AttributesFormatString=|
      | falling edges
      | active high
      mask Help: Output is active for one-cycle after each edge of the specified type (i.e. rising, falling, or both).  Latency is zero.
      mask TypeOptions edge: Rising | Falling | Both
      mask TypeOptions polarity: Active High | Active Low
      mask Display:
      | plot(x_in_num,0.5+y_in_num*0.2);
      | plot(x_out_num,0.5+y_out_num*0.2);
  pol1_in10_coeffs : Subsystem  AncestorBlock=casper_library_pfbs/pfb_coeff_gen  mask(pfb_coeff_gen){PFBSize=8, CoeffBitWidth=16, TotalTaps=8, CoeffDistMem=off, WindowType=hamming, bram_latency=2, n_inputs=4, nput=9, fwidth=1.245000000000000106581410364015, debug_mode=off, fan_latency=1}
      mask prompts: PFBSize "Size of PFB: (2^? pnts)"; CoeffBitWidth "Bitwidth of Coefficients:"; TotalTaps "Total Number of Taps:"; CoeffDistMem "Implement Coeff Gen in Distributed Memory"; WindowType "Windowing Function:"; bram_latency "BRAM Latency"; n_inputs "Number of Simultaneous Inputs: (2^?)"; nput "This is input number:"; fwidth "Bin Width (normal=1)"; debug_mode "Debug mode - coeffs are a [1:pfb_size*taps] ramp."; fan_latency "Fanout latency"
      mask init: same as rfsoc4x2_ospfb_128/pfb_fir_real10/pol1_in10_coeffs
      settings: AttributesFormatString=|
      | PFBSize=8, n_inputs=4,
      | taps=8, input=9
  pol1_in11_coeffs : Subsystem  AncestorBlock=casper_library_pfbs/pfb_coeff_gen  mask(pfb_coeff_gen){PFBSize=8, CoeffBitWidth=16, TotalTaps=8, CoeffDistMem=off, WindowType=hamming, bram_latency=2, n_inputs=4, nput=10, fwidth=1.245000000000000106581410364015, debug_mode=off, fan_latency=1}
      mask prompts: PFBSize "Size of PFB: (2^? pnts)"; CoeffBitWidth "Bitwidth of Coefficients:"; TotalTaps "Total Number of Taps:"; CoeffDistMem "Implement Coeff Gen in Distributed Memory"; WindowType "Windowing Function:"; bram_latency "BRAM Latency"; n_inputs "Number of Simultaneous Inputs: (2^?)"; nput "This is input number:"; fwidth "Bin Width (normal=1)"; debug_mode "Debug mode - coeffs are a [1:pfb_size*taps] ramp."; fan_latency "Fanout latency"
      mask init: same as rfsoc4x2_ospfb_128/pfb_fir_real10/pol1_in10_coeffs
      settings: AttributesFormatString=|
      | PFBSize=8, n_inputs=4,
      | taps=8, input=10
  pol1_in12_coeffs : Subsystem  AncestorBlock=casper_library_pfbs/pfb_coeff_gen  mask(pfb_coeff_gen){PFBSize=8, CoeffBitWidth=16, TotalTaps=8, CoeffDistMem=off, WindowType=hamming, bram_latency=2, n_inputs=4, nput=11, fwidth=1.245000000000000106581410364015, debug_mode=off, fan_latency=1}
      mask prompts: PFBSize "Size of PFB: (2^? pnts)"; CoeffBitWidth "Bitwidth of Coefficients:"; TotalTaps "Total Number of Taps:"; CoeffDistMem "Implement Coeff Gen in Distributed Memory"; WindowType "Windowing Function:"; bram_latency "BRAM Latency"; n_inputs "Number of Simultaneous Inputs: (2^?)"; nput "This is input number:"; fwidth "Bin Width (normal=1)"; debug_mode "Debug mode - coeffs are a [1:pfb_size*taps] ramp."; fan_latency "Fanout latency"
      mask init: same as rfsoc4x2_ospfb_128/pfb_fir_real10/pol1_in10_coeffs
      settings: AttributesFormatString=|
      | PFBSize=8, n_inputs=4,
      | taps=8, input=11
  pol1_in13_coeffs : Subsystem  AncestorBlock=casper_library_pfbs/pfb_coeff_gen  mask(pfb_coeff_gen){PFBSize=8, CoeffBitWidth=16, TotalTaps=8, CoeffDistMem=off, WindowType=hamming, bram_latency=2, n_inputs=4, nput=12, fwidth=1.245000000000000106581410364015, debug_mode=off, fan_latency=1}
      mask prompts: PFBSize "Size of PFB: (2^? pnts)"; CoeffBitWidth "Bitwidth of Coefficients:"; TotalTaps "Total Number of Taps:"; CoeffDistMem "Implement Coeff Gen in Distributed Memory"; WindowType "Windowing Function:"; bram_latency "BRAM Latency"; n_inputs "Number of Simultaneous Inputs: (2^?)"; nput "This is input number:"; fwidth "Bin Width (normal=1)"; debug_mode "Debug mode - coeffs are a [1:pfb_size*taps] ramp."; fan_latency "Fanout latency"
      mask init: same as rfsoc4x2_ospfb_128/pfb_fir_real10/pol1_in10_coeffs
      settings: AttributesFormatString=|
      | PFBSize=8, n_inputs=4,
      | taps=8, input=12
  pol1_in14_coeffs : Subsystem  AncestorBlock=casper_library_pfbs/pfb_coeff_gen  mask(pfb_coeff_gen){PFBSize=8, CoeffBitWidth=16, TotalTaps=8, CoeffDistMem=off, WindowType=hamming, bram_latency=2, n_inputs=4, nput=13, fwidth=1.245000000000000106581410364015, debug_mode=off, fan_latency=1}
      mask prompts: PFBSize "Size of PFB: (2^? pnts)"; CoeffBitWidth "Bitwidth of Coefficients:"; TotalTaps "Total Number of Taps:"; CoeffDistMem "Implement Coeff Gen in Distributed Memory"; WindowType "Windowing Function:"; bram_latency "BRAM Latency"; n_inputs "Number of Simultaneous Inputs: (2^?)"; nput "This is input number:"; fwidth "Bin Width (normal=1)"; debug_mode "Debug mode - coeffs are a [1:pfb_size*taps] ramp."; fan_latency "Fanout latency"
      mask init: same as rfsoc4x2_ospfb_128/pfb_fir_real10/pol1_in10_coeffs
      settings: AttributesFormatString=|
      | PFBSize=8, n_inputs=4,
      | taps=8, input=13
  pol1_in15_coeffs : Subsystem  AncestorBlock=casper_library_pfbs/pfb_coeff_gen  mask(pfb_coeff_gen){PFBSize=8, CoeffBitWidth=16, TotalTaps=8, CoeffDistMem=off, WindowType=hamming, bram_latency=2, n_inputs=4, nput=14, fwidth=1.245000000000000106581410364015, debug_mode=off, fan_latency=1}
      mask prompts: PFBSize "Size of PFB: (2^? pnts)"; CoeffBitWidth "Bitwidth of Coefficients:"; TotalTaps "Total Number of Taps:"; CoeffDistMem "Implement Coeff Gen in Distributed Memory"; WindowType "Windowing Function:"; bram_latency "BRAM Latency"; n_inputs "Number of Simultaneous Inputs: (2^?)"; nput "This is input number:"; fwidth "Bin Width (normal=1)"; debug_mode "Debug mode - coeffs are a [1:pfb_size*taps] ramp."; fan_latency "Fanout latency"
      mask init: same as rfsoc4x2_ospfb_128/pfb_fir_real10/pol1_in10_coeffs
      settings: AttributesFormatString=|
      | PFBSize=8, n_inputs=4,
      | taps=8, input=14
  pol1_in16_coeffs : Subsystem  AncestorBlock=casper_library_pfbs/pfb_coeff_gen  mask(pfb_coeff_gen){PFBSize=8, CoeffBitWidth=16, TotalTaps=8, CoeffDistMem=off, WindowType=hamming, bram_latency=2, n_inputs=4, nput=15, fwidth=1.245000000000000106581410364015, debug_mode=off, fan_latency=1}
      mask prompts: PFBSize "Size of PFB: (2^? pnts)"; CoeffBitWidth "Bitwidth of Coefficients:"; TotalTaps "Total Number of Taps:"; CoeffDistMem "Implement Coeff Gen in Distributed Memory"; WindowType "Windowing Function:"; bram_latency "BRAM Latency"; n_inputs "Number of Simultaneous Inputs: (2^?)"; nput "This is input number:"; fwidth "Bin Width (normal=1)"; debug_mode "Debug mode - coeffs are a [1:pfb_size*taps] ramp."; fan_latency "Fanout latency"
      mask init: same as rfsoc4x2_ospfb_128/pfb_fir_real10/pol1_in10_coeffs
      settings: AttributesFormatString=|
      | PFBSize=8, n_inputs=4,
      | taps=8, input=15
  pol1_in1_coeffs : Subsystem  AncestorBlock=casper_library_pfbs/pfb_coeff_gen  mask(pfb_coeff_gen){PFBSize=8, CoeffBitWidth=16, TotalTaps=8, CoeffDistMem=off, WindowType=hamming, bram_latency=2, n_inputs=4, nput=0, fwidth=1.245000000000000106581410364015, debug_mode=off, fan_latency=1}
      mask prompts: PFBSize "Size of PFB: (2^? pnts)"; CoeffBitWidth "Bitwidth of Coefficients:"; TotalTaps "Total Number of Taps:"; CoeffDistMem "Implement Coeff Gen in Distributed Memory"; WindowType "Windowing Function:"; bram_latency "BRAM Latency"; n_inputs "Number of Simultaneous Inputs: (2^?)"; nput "This is input number:"; fwidth "Bin Width (normal=1)"; debug_mode "Debug mode - coeffs are a [1:pfb_size*taps] ramp."; fan_latency "Fanout latency"
      mask init: same as rfsoc4x2_ospfb_128/pfb_fir_real10/pol1_in10_coeffs
      settings: AttributesFormatString=|
      | PFBSize=8, n_inputs=4,
      | taps=8, input=0
  pol1_in1_first_tap : Subsystem  AncestorBlock=casper_library_pfbs/first_tap_real  mask(first_tap_real){PFBSize=8, n_pol_blocks=1, CoeffBitWidth=16, TotalTaps=8, BitWidthIn=16, WindowType=hamming, mult_latency=2, bram_latency=2, n_inputs=4, fwidth=1.245000000000000106581410364015, use_hdl=on, use_embedded=off}
      mask prompts: PFBSize "Size of PFB: (2^? pnts)"; n_pol_blocks "Number of serial polarization blocks"; CoeffBitWidth "Bitwidth of Coefficients:"; TotalTaps "Total Number of Taps:"; BitWidthIn "Input Bitwidth:"; WindowType "Windowing Function:"; mult_latency "Mult Latency"; bram_latency "BRAM Latency"; n_inputs "Number of Simultaneous Inputs: (2^?)"; fwidth "Bit Width (normal=1)"; use_hdl "Use behavioral HDL for multlipliers"; use_embedded "Use embedded multipliers"
      mask init: same as rfsoc4x2_ospfb_128/pfb_fir_real10/pol1_in1_first_tap
      settings: AttributesFormatString=taps=8
      mask TypeOptions WindowType: bartlett | barthannwin | blackman | blackmanharris | bohamwin | chebwin | flattopwin | gausswin | hamming | hann | kaiser | nuttallwin | parzenwin | rectwin | tukeywin | triang | userwindow
      mask Callback use_hdl:
      | use_hdl = get_param(gcb,'use_hdl');
      | if( strcmp(use_hdl,'on')),
      |     set_param(gcb, 'use_embedded','off');
      |     set_param(gcb, 'MaskVisibilities',{'on','on','on','on','on','on','on','on','on','on','on','off'});
      | else,
      |     set_param(gcb, 'MaskVisibilities',{'on','on','on','on','on','on','on','on','on','on','on','on'});
      | end
  pol1_in1_first_tap1 : Subsystem  AncestorBlock=casper_library_pfbs/first_tap_real  mask(first_tap_real){PFBSize=8, n_pol_blocks=1, CoeffBitWidth=16, TotalTaps=8, BitWidthIn=16, WindowType=hamming, mult_latency=2, bram_latency=2, n_inputs=4, fwidth=1.245000000000000106581410364015, use_hdl=on, use_embedded=off}
      mask prompts: PFBSize "Size of PFB: (2^? pnts)"; n_pol_blocks "Number of serial polarization blocks"; CoeffBitWidth "Bitwidth of Coefficients:"; TotalTaps "Total Number of Taps:"; BitWidthIn "Input Bitwidth:"; WindowType "Windowing Function:"; mult_latency "Mult Latency"; bram_latency "BRAM Latency"; n_inputs "Number of Simultaneous Inputs: (2^?)"; fwidth "Bit Width (normal=1)"; use_hdl "Use behavioral HDL for multlipliers"; use_embedded "Use embedded multipliers"
      mask init: same as rfsoc4x2_ospfb_128/pfb_fir_real10/pol1_in1_first_tap
      settings: AttributesFormatString=taps=8
      mask TypeOptions WindowType: bartlett | barthannwin | blackman | blackmanharris | bohamwin | chebwin | flattopwin | gausswin | hamming | hann | kaiser | nuttallwin | parzenwin | rectwin | tukeywin | triang | userwindow
      mask Callback use_hdl:
      | use_hdl = get_param(gcb,'use_hdl');
      | if( strcmp(use_hdl,'on')),
      |     set_param(gcb, 'use_embedded','off');
      |     set_param(gcb, 'MaskVisibilities',{'on','on','on','on','on','on','on','on','on','on','on','off'});
      | else,
      |     set_param(gcb, 'MaskVisibilities',{'on','on','on','on','on','on','on','on','on','on','on','on'});
      | end
  pol1_in1_first_tap10 : Subsystem  AncestorBlock=casper_library_pfbs/first_tap_real  mask(first_tap_real){PFBSize=8, n_pol_blocks=1, CoeffBitWidth=16, TotalTaps=8, BitWidthIn=16, WindowType=hamming, mult_latency=2, bram_latency=2, n_inputs=4, fwidth=1.245000000000000106581410364015, use_hdl=on, use_embedded=off}
      mask prompts: PFBSize "Size of PFB: (2^? pnts)"; n_pol_blocks "Number of serial polarization blocks"; CoeffBitWidth "Bitwidth of Coefficients:"; TotalTaps "Total Number of Taps:"; BitWidthIn "Input Bitwidth:"; WindowType "Windowing Function:"; mult_latency "Mult Latency"; bram_latency "BRAM Latency"; n_inputs "Number of Simultaneous Inputs: (2^?)"; fwidth "Bit Width (normal=1)"; use_hdl "Use behavioral HDL for multlipliers"; use_embedded "Use embedded multipliers"
      mask init: same as rfsoc4x2_ospfb_128/pfb_fir_real10/pol1_in1_first_tap
      settings: AttributesFormatString=taps=8
      mask TypeOptions WindowType: bartlett | barthannwin | blackman | blackmanharris | bohamwin | chebwin | flattopwin | gausswin | hamming | hann | kaiser | nuttallwin | parzenwin | rectwin | tukeywin | triang | userwindow
      mask Callback use_hdl:
      | use_hdl = get_param(gcb,'use_hdl');
      | if( strcmp(use_hdl,'on')),
      |     set_param(gcb, 'use_embedded','off');
      |     set_param(gcb, 'MaskVisibilities',{'on','on','on','on','on','on','on','on','on','on','on','off'});
      | else,
      |     set_param(gcb, 'MaskVisibilities',{'on','on','on','on','on','on','on','on','on','on','on','on'});
      | end
  pol1_in1_first_tap11 : Subsystem  AncestorBlock=casper_library_pfbs/first_tap_real  mask(first_tap_real){PFBSize=8, n_pol_blocks=1, CoeffBitWidth=16, TotalTaps=8, BitWidthIn=16, WindowType=hamming, mult_latency=2, bram_latency=2, n_inputs=4, fwidth=1.245000000000000106581410364015, use_hdl=on, use_embedded=off}
      mask prompts: PFBSize "Size of PFB: (2^? pnts)"; n_pol_blocks "Number of serial polarization blocks"; CoeffBitWidth "Bitwidth of Coefficients:"; TotalTaps "Total Number of Taps:"; BitWidthIn "Input Bitwidth:"; WindowType "Windowing Function:"; mult_latency "Mult Latency"; bram_latency "BRAM Latency"; n_inputs "Number of Simultaneous Inputs: (2^?)"; fwidth "Bit Width (normal=1)"; use_hdl "Use behavioral HDL for multlipliers"; use_embedded "Use embedded multipliers"
      mask init: same as rfsoc4x2_ospfb_128/pfb_fir_real10/pol1_in1_first_tap
      settings: AttributesFormatString=taps=8
      mask TypeOptions WindowType: bartlett | barthannwin | blackman | blackmanharris | bohamwin | chebwin | flattopwin | gausswin | hamming | hann | kaiser | nuttallwin | parzenwin | rectwin | tukeywin | triang | userwindow
      mask Callback use_hdl:
      | use_hdl = get_param(gcb,'use_hdl');
      | if( strcmp(use_hdl,'on')),
      |     set_param(gcb, 'use_embedded','off');
      |     set_param(gcb, 'MaskVisibilities',{'on','on','on','on','on','on','on','on','on','on','on','off'});
      | else,
      |     set_param(gcb, 'MaskVisibilities',{'on','on','on','on','on','on','on','on','on','on','on','on'});
      | end
  pol1_in1_first_tap12 : Subsystem  AncestorBlock=casper_library_pfbs/first_tap_real  mask(first_tap_real){PFBSize=8, n_pol_blocks=1, CoeffBitWidth=16, TotalTaps=8, BitWidthIn=16, WindowType=hamming, mult_latency=2, bram_latency=2, n_inputs=4, fwidth=1.245000000000000106581410364015, use_hdl=on, use_embedded=off}
      mask prompts: PFBSize "Size of PFB: (2^? pnts)"; n_pol_blocks "Number of serial polarization blocks"; CoeffBitWidth "Bitwidth of Coefficients:"; TotalTaps "Total Number of Taps:"; BitWidthIn "Input Bitwidth:"; WindowType "Windowing Function:"; mult_latency "Mult Latency"; bram_latency "BRAM Latency"; n_inputs "Number of Simultaneous Inputs: (2^?)"; fwidth "Bit Width (normal=1)"; use_hdl "Use behavioral HDL for multlipliers"; use_embedded "Use embedded multipliers"
      mask init: same as rfsoc4x2_ospfb_128/pfb_fir_real10/pol1_in1_first_tap
      settings: AttributesFormatString=taps=8
      mask TypeOptions WindowType: bartlett | barthannwin | blackman | blackmanharris | bohamwin | chebwin | flattopwin | gausswin | hamming | hann | kaiser | nuttallwin | parzenwin | rectwin | tukeywin | triang | userwindow
      mask Callback use_hdl:
      | use_hdl = get_param(gcb,'use_hdl');
      | if( strcmp(use_hdl,'on')),
      |     set_param(gcb, 'use_embedded','off');
      |     set_param(gcb, 'MaskVisibilities',{'on','on','on','on','on','on','on','on','on','on','on','off'});
      | else,
      |     set_param(gcb, 'MaskVisibilities',{'on','on','on','on','on','on','on','on','on','on','on','on'});
      | end
  pol1_in1_first_tap13 : Subsystem  AncestorBlock=casper_library_pfbs/first_tap_real  mask(first_tap_real){PFBSize=8, n_pol_blocks=1, CoeffBitWidth=16, TotalTaps=8, BitWidthIn=16, WindowType=hamming, mult_latency=2, bram_latency=2, n_inputs=4, fwidth=1.245000000000000106581410364015, use_hdl=on, use_embedded=off}
      mask prompts: PFBSize "Size of PFB: (2^? pnts)"; n_pol_blocks "Number of serial polarization blocks"; CoeffBitWidth "Bitwidth of Coefficients:"; TotalTaps "Total Number of Taps:"; BitWidthIn "Input Bitwidth:"; WindowType "Windowing Function:"; mult_latency "Mult Latency"; bram_latency "BRAM Latency"; n_inputs "Number of Simultaneous Inputs: (2^?)"; fwidth "Bit Width (normal=1)"; use_hdl "Use behavioral HDL for multlipliers"; use_embedded "Use embedded multipliers"
      mask init: same as rfsoc4x2_ospfb_128/pfb_fir_real10/pol1_in1_first_tap
      settings: AttributesFormatString=taps=8
      mask TypeOptions WindowType: bartlett | barthannwin | blackman | blackmanharris | bohamwin | chebwin | flattopwin | gausswin | hamming | hann | kaiser | nuttallwin | parzenwin | rectwin | tukeywin | triang | userwindow
      mask Callback use_hdl:
      | use_hdl = get_param(gcb,'use_hdl');
      | if( strcmp(use_hdl,'on')),
      |     set_param(gcb, 'use_embedded','off');
      |     set_param(gcb, 'MaskVisibilities',{'on','on','on','on','on','on','on','on','on','on','on','off'});
      | else,
      |     set_param(gcb, 'MaskVisibilities',{'on','on','on','on','on','on','on','on','on','on','on','on'});
      | end
  pol1_in1_first_tap14 : Subsystem  AncestorBlock=casper_library_pfbs/first_tap_real  mask(first_tap_real){PFBSize=8, n_pol_blocks=1, CoeffBitWidth=16, TotalTaps=8, BitWidthIn=16, WindowType=hamming, mult_latency=2, bram_latency=2, n_inputs=4, fwidth=1.245000000000000106581410364015, use_hdl=on, use_embedded=off}
      mask prompts: PFBSize "Size of PFB: (2^? pnts)"; n_pol_blocks "Number of serial polarization blocks"; CoeffBitWidth "Bitwidth of Coefficients:"; TotalTaps "Total Number of Taps:"; BitWidthIn "Input Bitwidth:"; WindowType "Windowing Function:"; mult_latency "Mult Latency"; bram_latency "BRAM Latency"; n_inputs "Number of Simultaneous Inputs: (2^?)"; fwidth "Bit Width (normal=1)"; use_hdl "Use behavioral HDL for multlipliers"; use_embedded "Use embedded multipliers"
      mask init: same as rfsoc4x2_ospfb_128/pfb_fir_real10/pol1_in1_first_tap
      settings: AttributesFormatString=taps=8
      mask TypeOptions WindowType: bartlett | barthannwin | blackman | blackmanharris | bohamwin | chebwin | flattopwin | gausswin | hamming | hann | kaiser | nuttallwin | parzenwin | rectwin | tukeywin | triang | userwindow
      mask Callback use_hdl:
      | use_hdl = get_param(gcb,'use_hdl');
      | if( strcmp(use_hdl,'on')),
      |     set_param(gcb, 'use_embedded','off');
      |     set_param(gcb, 'MaskVisibilities',{'on','on','on','on','on','on','on','on','on','on','on','off'});
      | else,
      |     set_param(gcb, 'MaskVisibilities',{'on','on','on','on','on','on','on','on','on','on','on','on'});
      | end
  pol1_in1_first_tap15 : Subsystem  AncestorBlock=casper_library_pfbs/first_tap_real  mask(first_tap_real){PFBSize=8, n_pol_blocks=1, CoeffBitWidth=16, TotalTaps=8, BitWidthIn=16, WindowType=hamming, mult_latency=2, bram_latency=2, n_inputs=4, fwidth=1.245000000000000106581410364015, use_hdl=on, use_embedded=off}
      mask prompts: PFBSize "Size of PFB: (2^? pnts)"; n_pol_blocks "Number of serial polarization blocks"; CoeffBitWidth "Bitwidth of Coefficients:"; TotalTaps "Total Number of Taps:"; BitWidthIn "Input Bitwidth:"; WindowType "Windowing Function:"; mult_latency "Mult Latency"; bram_latency "BRAM Latency"; n_inputs "Number of Simultaneous Inputs: (2^?)"; fwidth "Bit Width (normal=1)"; use_hdl "Use behavioral HDL for multlipliers"; use_embedded "Use embedded multipliers"
      mask init: same as rfsoc4x2_ospfb_128/pfb_fir_real10/pol1_in1_first_tap
      settings: AttributesFormatString=taps=8
      mask TypeOptions WindowType: bartlett | barthannwin | blackman | blackmanharris | bohamwin | chebwin | flattopwin | gausswin | hamming | hann | kaiser | nuttallwin | parzenwin | rectwin | tukeywin | triang | userwindow
      mask Callback use_hdl:
      | use_hdl = get_param(gcb,'use_hdl');
      | if( strcmp(use_hdl,'on')),
      |     set_param(gcb, 'use_embedded','off');
      |     set_param(gcb, 'MaskVisibilities',{'on','on','on','on','on','on','on','on','on','on','on','off'});
      | else,
      |     set_param(gcb, 'MaskVisibilities',{'on','on','on','on','on','on','on','on','on','on','on','on'});
      | end
  pol1_in1_first_tap2 : Subsystem  AncestorBlock=casper_library_pfbs/first_tap_real  mask(first_tap_real){PFBSize=8, n_pol_blocks=1, CoeffBitWidth=16, TotalTaps=8, BitWidthIn=16, WindowType=hamming, mult_latency=2, bram_latency=2, n_inputs=4, fwidth=1.245000000000000106581410364015, use_hdl=on, use_embedded=off}
      mask prompts: PFBSize "Size of PFB: (2^? pnts)"; n_pol_blocks "Number of serial polarization blocks"; CoeffBitWidth "Bitwidth of Coefficients:"; TotalTaps "Total Number of Taps:"; BitWidthIn "Input Bitwidth:"; WindowType "Windowing Function:"; mult_latency "Mult Latency"; bram_latency "BRAM Latency"; n_inputs "Number of Simultaneous Inputs: (2^?)"; fwidth "Bit Width (normal=1)"; use_hdl "Use behavioral HDL for multlipliers"; use_embedded "Use embedded multipliers"
      mask init: same as rfsoc4x2_ospfb_128/pfb_fir_real10/pol1_in1_first_tap
      settings: AttributesFormatString=taps=8
      mask TypeOptions WindowType: bartlett | barthannwin | blackman | blackmanharris | bohamwin | chebwin | flattopwin | gausswin | hamming | hann | kaiser | nuttallwin | parzenwin | rectwin | tukeywin | triang | userwindow
      mask Callback use_hdl:
      | use_hdl = get_param(gcb,'use_hdl');
      | if( strcmp(use_hdl,'on')),
      |     set_param(gcb, 'use_embedded','off');
      |     set_param(gcb, 'MaskVisibilities',{'on','on','on','on','on','on','on','on','on','on','on','off'});
      | else,
      |     set_param(gcb, 'MaskVisibilities',{'on','on','on','on','on','on','on','on','on','on','on','on'});
      | end
  pol1_in1_first_tap3 : Subsystem  AncestorBlock=casper_library_pfbs/first_tap_real  mask(first_tap_real){PFBSize=8, n_pol_blocks=1, CoeffBitWidth=16, TotalTaps=8, BitWidthIn=16, WindowType=hamming, mult_latency=2, bram_latency=2, n_inputs=4, fwidth=1.245000000000000106581410364015, use_hdl=on, use_embedded=off}
      mask prompts: PFBSize "Size of PFB: (2^? pnts)"; n_pol_blocks "Number of serial polarization blocks"; CoeffBitWidth "Bitwidth of Coefficients:"; TotalTaps "Total Number of Taps:"; BitWidthIn "Input Bitwidth:"; WindowType "Windowing Function:"; mult_latency "Mult Latency"; bram_latency "BRAM Latency"; n_inputs "Number of Simultaneous Inputs: (2^?)"; fwidth "Bit Width (normal=1)"; use_hdl "Use behavioral HDL for multlipliers"; use_embedded "Use embedded multipliers"
      mask init: same as rfsoc4x2_ospfb_128/pfb_fir_real10/pol1_in1_first_tap
      settings: AttributesFormatString=taps=8
      mask TypeOptions WindowType: bartlett | barthannwin | blackman | blackmanharris | bohamwin | chebwin | flattopwin | gausswin | hamming | hann | kaiser | nuttallwin | parzenwin | rectwin | tukeywin | triang | userwindow
      mask Callback use_hdl:
      | use_hdl = get_param(gcb,'use_hdl');
      | if( strcmp(use_hdl,'on')),
      |     set_param(gcb, 'use_embedded','off');
      |     set_param(gcb, 'MaskVisibilities',{'on','on','on','on','on','on','on','on','on','on','on','off'});
      | else,
      |     set_param(gcb, 'MaskVisibilities',{'on','on','on','on','on','on','on','on','on','on','on','on'});
      | end
  pol1_in1_first_tap4 : Subsystem  AncestorBlock=casper_library_pfbs/first_tap_real  mask(first_tap_real){PFBSize=8, n_pol_blocks=1, CoeffBitWidth=16, TotalTaps=8, BitWidthIn=16, WindowType=hamming, mult_latency=2, bram_latency=2, n_inputs=4, fwidth=1.245000000000000106581410364015, use_hdl=on, use_embedded=off}
      mask prompts: PFBSize "Size of PFB: (2^? pnts)"; n_pol_blocks "Number of serial polarization blocks"; CoeffBitWidth "Bitwidth of Coefficients:"; TotalTaps "Total Number of Taps:"; BitWidthIn "Input Bitwidth:"; WindowType "Windowing Function:"; mult_latency "Mult Latency"; bram_latency "BRAM Latency"; n_inputs "Number of Simultaneous Inputs: (2^?)"; fwidth "Bit Width (normal=1)"; use_hdl "Use behavioral HDL for multlipliers"; use_embedded "Use embedded multipliers"
      mask init: same as rfsoc4x2_ospfb_128/pfb_fir_real10/pol1_in1_first_tap
      settings: AttributesFormatString=taps=8
      mask TypeOptions WindowType: bartlett | barthannwin | blackman | blackmanharris | bohamwin | chebwin | flattopwin | gausswin | hamming | hann | kaiser | nuttallwin | parzenwin | rectwin | tukeywin | triang | userwindow
      mask Callback use_hdl:
      | use_hdl = get_param(gcb,'use_hdl');
      | if( strcmp(use_hdl,'on')),
      |     set_param(gcb, 'use_embedded','off');
      |     set_param(gcb, 'MaskVisibilities',{'on','on','on','on','on','on','on','on','on','on','on','off'});
      | else,
      |     set_param(gcb, 'MaskVisibilities',{'on','on','on','on','on','on','on','on','on','on','on','on'});
      | end
  pol1_in1_first_tap5 : Subsystem  AncestorBlock=casper_library_pfbs/first_tap_real  mask(first_tap_real){PFBSize=8, n_pol_blocks=1, CoeffBitWidth=16, TotalTaps=8, BitWidthIn=16, WindowType=hamming, mult_latency=2, bram_latency=2, n_inputs=4, fwidth=1.245000000000000106581410364015, use_hdl=on, use_embedded=off}
      mask prompts: PFBSize "Size of PFB: (2^? pnts)"; n_pol_blocks "Number of serial polarization blocks"; CoeffBitWidth "Bitwidth of Coefficients:"; TotalTaps "Total Number of Taps:"; BitWidthIn "Input Bitwidth:"; WindowType "Windowing Function:"; mult_latency "Mult Latency"; bram_latency "BRAM Latency"; n_inputs "Number of Simultaneous Inputs: (2^?)"; fwidth "Bit Width (normal=1)"; use_hdl "Use behavioral HDL for multlipliers"; use_embedded "Use embedded multipliers"
      mask init: same as rfsoc4x2_ospfb_128/pfb_fir_real10/pol1_in1_first_tap
      settings: AttributesFormatString=taps=8
      mask TypeOptions WindowType: bartlett | barthannwin | blackman | blackmanharris | bohamwin | chebwin | flattopwin | gausswin | hamming | hann | kaiser | nuttallwin | parzenwin | rectwin | tukeywin | triang | userwindow
      mask Callback use_hdl:
      | use_hdl = get_param(gcb,'use_hdl');
      | if( strcmp(use_hdl,'on')),
      |     set_param(gcb, 'use_embedded','off');
      |     set_param(gcb, 'MaskVisibilities',{'on','on','on','on','on','on','on','on','on','on','on','off'});
      | else,
      |     set_param(gcb, 'MaskVisibilities',{'on','on','on','on','on','on','on','on','on','on','on','on'});
      | end
  pol1_in1_first_tap6 : Subsystem  AncestorBlock=casper_library_pfbs/first_tap_real  mask(first_tap_real){PFBSize=8, n_pol_blocks=1, CoeffBitWidth=16, TotalTaps=8, BitWidthIn=16, WindowType=hamming, mult_latency=2, bram_latency=2, n_inputs=4, fwidth=1.245000000000000106581410364015, use_hdl=on, use_embedded=off}
      mask prompts: PFBSize "Size of PFB: (2^? pnts)"; n_pol_blocks "Number of serial polarization blocks"; CoeffBitWidth "Bitwidth of Coefficients:"; TotalTaps "Total Number of Taps:"; BitWidthIn "Input Bitwidth:"; WindowType "Windowing Function:"; mult_latency "Mult Latency"; bram_latency "BRAM Latency"; n_inputs "Number of Simultaneous Inputs: (2^?)"; fwidth "Bit Width (normal=1)"; use_hdl "Use behavioral HDL for multlipliers"; use_embedded "Use embedded multipliers"
      mask init: same as rfsoc4x2_ospfb_128/pfb_fir_real10/pol1_in1_first_tap
      settings: AttributesFormatString=taps=8
      mask TypeOptions WindowType: bartlett | barthannwin | blackman | blackmanharris | bohamwin | chebwin | flattopwin | gausswin | hamming | hann | kaiser | nuttallwin | parzenwin | rectwin | tukeywin | triang | userwindow
      mask Callback use_hdl:
      | use_hdl = get_param(gcb,'use_hdl');
      | if( strcmp(use_hdl,'on')),
      |     set_param(gcb, 'use_embedded','off');
      |     set_param(gcb, 'MaskVisibilities',{'on','on','on','on','on','on','on','on','on','on','on','off'});
      | else,
      |     set_param(gcb, 'MaskVisibilities',{'on','on','on','on','on','on','on','on','on','on','on','on'});
      | end
  pol1_in1_first_tap7 : Subsystem  AncestorBlock=casper_library_pfbs/first_tap_real  mask(first_tap_real){PFBSize=8, n_pol_blocks=1, CoeffBitWidth=16, TotalTaps=8, BitWidthIn=16, WindowType=hamming, mult_latency=2, bram_latency=2, n_inputs=4, fwidth=1.245000000000000106581410364015, use_hdl=on, use_embedded=off}
      mask prompts: PFBSize "Size of PFB: (2^? pnts)"; n_pol_blocks "Number of serial polarization blocks"; CoeffBitWidth "Bitwidth of Coefficients:"; TotalTaps "Total Number of Taps:"; BitWidthIn "Input Bitwidth:"; WindowType "Windowing Function:"; mult_latency "Mult Latency"; bram_latency "BRAM Latency"; n_inputs "Number of Simultaneous Inputs: (2^?)"; fwidth "Bit Width (normal=1)"; use_hdl "Use behavioral HDL for multlipliers"; use_embedded "Use embedded multipliers"
      mask init: same as rfsoc4x2_ospfb_128/pfb_fir_real10/pol1_in1_first_tap
      settings: AttributesFormatString=taps=8
      mask TypeOptions WindowType: bartlett | barthannwin | blackman | blackmanharris | bohamwin | chebwin | flattopwin | gausswin | hamming | hann | kaiser | nuttallwin | parzenwin | rectwin | tukeywin | triang | userwindow
      mask Callback use_hdl:
      | use_hdl = get_param(gcb,'use_hdl');
      | if( strcmp(use_hdl,'on')),
      |     set_param(gcb, 'use_embedded','off');
      |     set_param(gcb, 'MaskVisibilities',{'on','on','on','on','on','on','on','on','on','on','on','off'});
      | else,
      |     set_param(gcb, 'MaskVisibilities',{'on','on','on','on','on','on','on','on','on','on','on','on'});
      | end
  pol1_in1_first_tap8 : Subsystem  AncestorBlock=casper_library_pfbs/first_tap_real  mask(first_tap_real){PFBSize=8, n_pol_blocks=1, CoeffBitWidth=16, TotalTaps=8, BitWidthIn=16, WindowType=hamming, mult_latency=2, bram_latency=2, n_inputs=4, fwidth=1.245000000000000106581410364015, use_hdl=on, use_embedded=off}
      mask prompts: PFBSize "Size of PFB: (2^? pnts)"; n_pol_blocks "Number of serial polarization blocks"; CoeffBitWidth "Bitwidth of Coefficients:"; TotalTaps "Total Number of Taps:"; BitWidthIn "Input Bitwidth:"; WindowType "Windowing Function:"; mult_latency "Mult Latency"; bram_latency "BRAM Latency"; n_inputs "Number of Simultaneous Inputs: (2^?)"; fwidth "Bit Width (normal=1)"; use_hdl "Use behavioral HDL for multlipliers"; use_embedded "Use embedded multipliers"
      mask init: same as rfsoc4x2_ospfb_128/pfb_fir_real10/pol1_in1_first_tap
      settings: AttributesFormatString=taps=8
      mask TypeOptions WindowType: bartlett | barthannwin | blackman | blackmanharris | bohamwin | chebwin | flattopwin | gausswin | hamming | hann | kaiser | nuttallwin | parzenwin | rectwin | tukeywin | triang | userwindow
      mask Callback use_hdl:
      | use_hdl = get_param(gcb,'use_hdl');
      | if( strcmp(use_hdl,'on')),
      |     set_param(gcb, 'use_embedded','off');
      |     set_param(gcb, 'MaskVisibilities',{'on','on','on','on','on','on','on','on','on','on','on','off'});
      | else,
      |     set_param(gcb, 'MaskVisibilities',{'on','on','on','on','on','on','on','on','on','on','on','on'});
      | end
  pol1_in1_first_tap9 : Subsystem  AncestorBlock=casper_library_pfbs/first_tap_real  mask(first_tap_real){PFBSize=8, n_pol_blocks=1, CoeffBitWidth=16, TotalTaps=8, BitWidthIn=16, WindowType=hamming, mult_latency=2, bram_latency=2, n_inputs=4, fwidth=1.245000000000000106581410364015, use_hdl=on, use_embedded=off}
      mask prompts: PFBSize "Size of PFB: (2^? pnts)"; n_pol_blocks "Number of serial polarization blocks"; CoeffBitWidth "Bitwidth of Coefficients:"; TotalTaps "Total Number of Taps:"; BitWidthIn "Input Bitwidth:"; WindowType "Windowing Function:"; mult_latency "Mult Latency"; bram_latency "BRAM Latency"; n_inputs "Number of Simultaneous Inputs: (2^?)"; fwidth "Bit Width (normal=1)"; use_hdl "Use behavioral HDL for multlipliers"; use_embedded "Use embedded multipliers"
      mask init: same as rfsoc4x2_ospfb_128/pfb_fir_real10/pol1_in1_first_tap
      settings: AttributesFormatString=taps=8
      mask TypeOptions WindowType: bartlett | barthannwin | blackman | blackmanharris | bohamwin | chebwin | flattopwin | gausswin | hamming | hann | kaiser | nuttallwin | parzenwin | rectwin | tukeywin | triang | userwindow
      mask Callback use_hdl:
      | use_hdl = get_param(gcb,'use_hdl');
      | if( strcmp(use_hdl,'on')),
      |     set_param(gcb, 'use_embedded','off');
      |     set_param(gcb, 'MaskVisibilities',{'on','on','on','on','on','on','on','on','on','on','on','off'});
      | else,
      |     set_param(gcb, 'MaskVisibilities',{'on','on','on','on','on','on','on','on','on','on','on','on'});
      | end
  pol1_in1_last_tap : Subsystem  AncestorBlock=casper_library_pfbs/last_tap_real  mask(last_tap_real){BitWidthIn=16, CoeffBitWidth=16, mult_latency=2, use_hdl=on, use_embedded=off}
      mask prompts: BitWidthIn "Input Bitwidth:"; CoeffBitWidth "Coeff Bitwidth:"; mult_latency "Mult Latency"; use_hdl "Use behavioral HDL for multlipliers"; use_embedded "Use embedded multipliers"
      mask init:
      | last_tap_real_init(gcb,...
      |     'BitWidthIn', BitWidthIn,...
      |     'CoeffBitWidth', CoeffBitWidth,...
      |     'mult_latency', mult_latency,...
      |     'use_hdl', use_hdl,...
      |     'use_embedded', use_embedded);
      mask Callback use_hdl:
      | use_hdl = get_param(gcb,'use_hdl');
      | if( strcmp(use_hdl,'on')),
      |     set_param(gcb, 'use_embedded','off');
      |     set_param(gcb, 'MaskVisibilities',{'on','on','on','on','off'});
      | else,
      |     set_param(gcb, 'MaskVisibilities',{'on','on','on','on','on'});
      | end
  pol1_in1_last_tap1 : Subsystem  AncestorBlock=casper_library_pfbs/last_tap_real  mask(last_tap_real){BitWidthIn=16, CoeffBitWidth=16, mult_latency=2, use_hdl=on, use_embedded=off}
      mask prompts: BitWidthIn "Input Bitwidth:"; CoeffBitWidth "Coeff Bitwidth:"; mult_latency "Mult Latency"; use_hdl "Use behavioral HDL for multlipliers"; use_embedded "Use embedded multipliers"
      mask init:
      | last_tap_real_init(gcb,...
      |     'BitWidthIn', BitWidthIn,...
      |     'CoeffBitWidth', CoeffBitWidth,...
      |     'mult_latency', mult_latency,...
      |     'use_hdl', use_hdl,...
      |     'use_embedded', use_embedded);
      mask Callback use_hdl:
      | use_hdl = get_param(gcb,'use_hdl');
      | if( strcmp(use_hdl,'on')),
      |     set_param(gcb, 'use_embedded','off');
      |     set_param(gcb, 'MaskVisibilities',{'on','on','on','on','off'});
      | else,
      |     set_param(gcb, 'MaskVisibilities',{'on','on','on','on','on'});
      | end
  pol1_in1_last_tap10 : Subsystem  AncestorBlock=casper_library_pfbs/last_tap_real  mask(last_tap_real){BitWidthIn=16, CoeffBitWidth=16, mult_latency=2, use_hdl=on, use_embedded=off}
      mask prompts: BitWidthIn "Input Bitwidth:"; CoeffBitWidth "Coeff Bitwidth:"; mult_latency "Mult Latency"; use_hdl "Use behavioral HDL for multlipliers"; use_embedded "Use embedded multipliers"
      mask init:
      | last_tap_real_init(gcb,...
      |     'BitWidthIn', BitWidthIn,...
      |     'CoeffBitWidth', CoeffBitWidth,...
      |     'mult_latency', mult_latency,...
      |     'use_hdl', use_hdl,...
      |     'use_embedded', use_embedded);
      mask Callback use_hdl:
      | use_hdl = get_param(gcb,'use_hdl');
      | if( strcmp(use_hdl,'on')),
      |     set_param(gcb, 'use_embedded','off');
      |     set_param(gcb, 'MaskVisibilities',{'on','on','on','on','off'});
      | else,
      |     set_param(gcb, 'MaskVisibilities',{'on','on','on','on','on'});
      | end
  pol1_in1_last_tap11 : Subsystem  AncestorBlock=casper_library_pfbs/last_tap_real  mask(last_tap_real){BitWidthIn=16, CoeffBitWidth=16, mult_latency=2, use_hdl=on, use_embedded=off}
      mask prompts: BitWidthIn "Input Bitwidth:"; CoeffBitWidth "Coeff Bitwidth:"; mult_latency "Mult Latency"; use_hdl "Use behavioral HDL for multlipliers"; use_embedded "Use embedded multipliers"
      mask init:
      | last_tap_real_init(gcb,...
      |     'BitWidthIn', BitWidthIn,...
      |     'CoeffBitWidth', CoeffBitWidth,...
      |     'mult_latency', mult_latency,...
      |     'use_hdl', use_hdl,...
      |     'use_embedded', use_embedded);
      mask Callback use_hdl:
      | use_hdl = get_param(gcb,'use_hdl');
      | if( strcmp(use_hdl,'on')),
      |     set_param(gcb, 'use_embedded','off');
      |     set_param(gcb, 'MaskVisibilities',{'on','on','on','on','off'});
      | else,
      |     set_param(gcb, 'MaskVisibilities',{'on','on','on','on','on'});
      | end
  pol1_in1_last_tap12 : Subsystem  AncestorBlock=casper_library_pfbs/last_tap_real  mask(last_tap_real){BitWidthIn=16, CoeffBitWidth=16, mult_latency=2, use_hdl=on, use_embedded=off}
      mask prompts: BitWidthIn "Input Bitwidth:"; CoeffBitWidth "Coeff Bitwidth:"; mult_latency "Mult Latency"; use_hdl "Use behavioral HDL for multlipliers"; use_embedded "Use embedded multipliers"
      mask init:
      | last_tap_real_init(gcb,...
      |     'BitWidthIn', BitWidthIn,...
      |     'CoeffBitWidth', CoeffBitWidth,...
      |     'mult_latency', mult_latency,...
      |     'use_hdl', use_hdl,...
      |     'use_embedded', use_embedded);
      mask Callback use_hdl:
      | use_hdl = get_param(gcb,'use_hdl');
      | if( strcmp(use_hdl,'on')),
      |     set_param(gcb, 'use_embedded','off');
      |     set_param(gcb, 'MaskVisibilities',{'on','on','on','on','off'});
      | else,
      |     set_param(gcb, 'MaskVisibilities',{'on','on','on','on','on'});
      | end
  pol1_in1_last_tap13 : Subsystem  AncestorBlock=casper_library_pfbs/last_tap_real  mask(last_tap_real){BitWidthIn=16, CoeffBitWidth=16, mult_latency=2, use_hdl=on, use_embedded=off}
      mask prompts: BitWidthIn "Input Bitwidth:"; CoeffBitWidth "Coeff Bitwidth:"; mult_latency "Mult Latency"; use_hdl "Use behavioral HDL for multlipliers"; use_embedded "Use embedded multipliers"
      mask init:
      | last_tap_real_init(gcb,...
      |     'BitWidthIn', BitWidthIn,...
      |     'CoeffBitWidth', CoeffBitWidth,...
      |     'mult_latency', mult_latency,...
      |     'use_hdl', use_hdl,...
      |     'use_embedded', use_embedded);
      mask Callback use_hdl:
      | use_hdl = get_param(gcb,'use_hdl');
      | if( strcmp(use_hdl,'on')),
      |     set_param(gcb, 'use_embedded','off');
      |     set_param(gcb, 'MaskVisibilities',{'on','on','on','on','off'});
      | else,
      |     set_param(gcb, 'MaskVisibilities',{'on','on','on','on','on'});
      | end
  pol1_in1_last_tap14 : Subsystem  AncestorBlock=casper_library_pfbs/last_tap_real  mask(last_tap_real){BitWidthIn=16, CoeffBitWidth=16, mult_latency=2, use_hdl=on, use_embedded=off}
      mask prompts: BitWidthIn "Input Bitwidth:"; CoeffBitWidth "Coeff Bitwidth:"; mult_latency "Mult Latency"; use_hdl "Use behavioral HDL for multlipliers"; use_embedded "Use embedded multipliers"
      mask init:
      | last_tap_real_init(gcb,...
      |     'BitWidthIn', BitWidthIn,...
      |     'CoeffBitWidth', CoeffBitWidth,...
      |     'mult_latency', mult_latency,...
      |     'use_hdl', use_hdl,...
      |     'use_embedded', use_embedded);
      mask Callback use_hdl:
      | use_hdl = get_param(gcb,'use_hdl');
      | if( strcmp(use_hdl,'on')),
      |     set_param(gcb, 'use_embedded','off');
      |     set_param(gcb, 'MaskVisibilities',{'on','on','on','on','off'});
      | else,
      |     set_param(gcb, 'MaskVisibilities',{'on','on','on','on','on'});
      | end
  pol1_in1_last_tap15 : Subsystem  AncestorBlock=casper_library_pfbs/last_tap_real  mask(last_tap_real){BitWidthIn=16, CoeffBitWidth=16, mult_latency=2, use_hdl=on, use_embedded=off}
      mask prompts: BitWidthIn "Input Bitwidth:"; CoeffBitWidth "Coeff Bitwidth:"; mult_latency "Mult Latency"; use_hdl "Use behavioral HDL for multlipliers"; use_embedded "Use embedded multipliers"
      mask init:
      | last_tap_real_init(gcb,...
      |     'BitWidthIn', BitWidthIn,...
      |     'CoeffBitWidth', CoeffBitWidth,...
      |     'mult_latency', mult_latency,...
      |     'use_hdl', use_hdl,...
      |     'use_embedded', use_embedded);
      mask Callback use_hdl:
      | use_hdl = get_param(gcb,'use_hdl');
      | if( strcmp(use_hdl,'on')),
      |     set_param(gcb, 'use_embedded','off');
      |     set_param(gcb, 'MaskVisibilities',{'on','on','on','on','off'});
      | else,
      |     set_param(gcb, 'MaskVisibilities',{'on','on','on','on','on'});
      | end
  pol1_in1_last_tap2 : Subsystem  AncestorBlock=casper_library_pfbs/last_tap_real  mask(last_tap_real){BitWidthIn=16, CoeffBitWidth=16, mult_latency=2, use_hdl=on, use_embedded=off}
      mask prompts: BitWidthIn "Input Bitwidth:"; CoeffBitWidth "Coeff Bitwidth:"; mult_latency "Mult Latency"; use_hdl "Use behavioral HDL for multlipliers"; use_embedded "Use embedded multipliers"
      mask init:
      | last_tap_real_init(gcb,...
      |     'BitWidthIn', BitWidthIn,...
      |     'CoeffBitWidth', CoeffBitWidth,...
      |     'mult_latency', mult_latency,...
      |     'use_hdl', use_hdl,...
      |     'use_embedded', use_embedded);
      mask Callback use_hdl:
      | use_hdl = get_param(gcb,'use_hdl');
      | if( strcmp(use_hdl,'on')),
      |     set_param(gcb, 'use_embedded','off');
      |     set_param(gcb, 'MaskVisibilities',{'on','on','on','on','off'});
      | else,
      |     set_param(gcb, 'MaskVisibilities',{'on','on','on','on','on'});
      | end
  pol1_in1_last_tap3 : Subsystem  AncestorBlock=casper_library_pfbs/last_tap_real  mask(last_tap_real){BitWidthIn=16, CoeffBitWidth=16, mult_latency=2, use_hdl=on, use_embedded=off}
      mask prompts: BitWidthIn "Input Bitwidth:"; CoeffBitWidth "Coeff Bitwidth:"; mult_latency "Mult Latency"; use_hdl "Use behavioral HDL for multlipliers"; use_embedded "Use embedded multipliers"
      mask init:
      | last_tap_real_init(gcb,...
      |     'BitWidthIn', BitWidthIn,...
      |     'CoeffBitWidth', CoeffBitWidth,...
      |     'mult_latency', mult_latency,...
      |     'use_hdl', use_hdl,...
      |     'use_embedded', use_embedded);
      mask Callback use_hdl:
      | use_hdl = get_param(gcb,'use_hdl');
      | if( strcmp(use_hdl,'on')),
      |     set_param(gcb, 'use_embedded','off');
      |     set_param(gcb, 'MaskVisibilities',{'on','on','on','on','off'});
      | else,
      |     set_param(gcb, 'MaskVisibilities',{'on','on','on','on','on'});
      | end
  pol1_in1_last_tap4 : Subsystem  AncestorBlock=casper_library_pfbs/last_tap_real  mask(last_tap_real){BitWidthIn=16, CoeffBitWidth=16, mult_latency=2, use_hdl=on, use_embedded=off}
      mask prompts: BitWidthIn "Input Bitwidth:"; CoeffBitWidth "Coeff Bitwidth:"; mult_latency "Mult Latency"; use_hdl "Use behavioral HDL for multlipliers"; use_embedded "Use embedded multipliers"
      mask init:
      | last_tap_real_init(gcb,...
      |     'BitWidthIn', BitWidthIn,...
      |     'CoeffBitWidth', CoeffBitWidth,...
      |     'mult_latency', mult_latency,...
      |     'use_hdl', use_hdl,...
      |     'use_embedded', use_embedded);
      mask Callback use_hdl:
      | use_hdl = get_param(gcb,'use_hdl');
      | if( strcmp(use_hdl,'on')),
      |     set_param(gcb, 'use_embedded','off');
      |     set_param(gcb, 'MaskVisibilities',{'on','on','on','on','off'});
      | else,
      |     set_param(gcb, 'MaskVisibilities',{'on','on','on','on','on'});
      | end
  pol1_in1_last_tap5 : Subsystem  AncestorBlock=casper_library_pfbs/last_tap_real  mask(last_tap_real){BitWidthIn=16, CoeffBitWidth=16, mult_latency=2, use_hdl=on, use_embedded=off}
      mask prompts: BitWidthIn "Input Bitwidth:"; CoeffBitWidth "Coeff Bitwidth:"; mult_latency "Mult Latency"; use_hdl "Use behavioral HDL for multlipliers"; use_embedded "Use embedded multipliers"
      mask init:
      | last_tap_real_init(gcb,...
      |     'BitWidthIn', BitWidthIn,...
      |     'CoeffBitWidth', CoeffBitWidth,...
      |     'mult_latency', mult_latency,...
      |     'use_hdl', use_hdl,...
      |     'use_embedded', use_embedded);
      mask Callback use_hdl:
      | use_hdl = get_param(gcb,'use_hdl');
      | if( strcmp(use_hdl,'on')),
      |     set_param(gcb, 'use_embedded','off');
      |     set_param(gcb, 'MaskVisibilities',{'on','on','on','on','off'});
      | else,
      |     set_param(gcb, 'MaskVisibilities',{'on','on','on','on','on'});
      | end
  pol1_in1_last_tap6 : Subsystem  AncestorBlock=casper_library_pfbs/last_tap_real  mask(last_tap_real){BitWidthIn=16, CoeffBitWidth=16, mult_latency=2, use_hdl=on, use_embedded=off}
      mask prompts: BitWidthIn "Input Bitwidth:"; CoeffBitWidth "Coeff Bitwidth:"; mult_latency "Mult Latency"; use_hdl "Use behavioral HDL for multlipliers"; use_embedded "Use embedded multipliers"
      mask init:
      | last_tap_real_init(gcb,...
      |     'BitWidthIn', BitWidthIn,...
      |     'CoeffBitWidth', CoeffBitWidth,...
      |     'mult_latency', mult_latency,...
      |     'use_hdl', use_hdl,...
      |     'use_embedded', use_embedded);
      mask Callback use_hdl:
      | use_hdl = get_param(gcb,'use_hdl');
      | if( strcmp(use_hdl,'on')),
      |     set_param(gcb, 'use_embedded','off');
      |     set_param(gcb, 'MaskVisibilities',{'on','on','on','on','off'});
      | else,
      |     set_param(gcb, 'MaskVisibilities',{'on','on','on','on','on'});
      | end
  pol1_in1_last_tap7 : Subsystem  AncestorBlock=casper_library_pfbs/last_tap_real  mask(last_tap_real){BitWidthIn=16, CoeffBitWidth=16, mult_latency=2, use_hdl=on, use_embedded=off}
      mask prompts: BitWidthIn "Input Bitwidth:"; CoeffBitWidth "Coeff Bitwidth:"; mult_latency "Mult Latency"; use_hdl "Use behavioral HDL for multlipliers"; use_embedded "Use embedded multipliers"
      mask init:
      | last_tap_real_init(gcb,...
      |     'BitWidthIn', BitWidthIn,...
      |     'CoeffBitWidth', CoeffBitWidth,...
      |     'mult_latency', mult_latency,...
      |     'use_hdl', use_hdl,...
      |     'use_embedded', use_embedded);
      mask Callback use_hdl:
      | use_hdl = get_param(gcb,'use_hdl');
      | if( strcmp(use_hdl,'on')),
      |     set_param(gcb, 'use_embedded','off');
      |     set_param(gcb, 'MaskVisibilities',{'on','on','on','on','off'});
      | else,
      |     set_param(gcb, 'MaskVisibilities',{'on','on','on','on','on'});
      | end
  pol1_in1_last_tap8 : Subsystem  AncestorBlock=casper_library_pfbs/last_tap_real  mask(last_tap_real){BitWidthIn=16, CoeffBitWidth=16, mult_latency=2, use_hdl=on, use_embedded=off}
      mask prompts: BitWidthIn "Input Bitwidth:"; CoeffBitWidth "Coeff Bitwidth:"; mult_latency "Mult Latency"; use_hdl "Use behavioral HDL for multlipliers"; use_embedded "Use embedded multipliers"
      mask init:
      | last_tap_real_init(gcb,...
      |     'BitWidthIn', BitWidthIn,...
      |     'CoeffBitWidth', CoeffBitWidth,...
      |     'mult_latency', mult_latency,...
      |     'use_hdl', use_hdl,...
      |     'use_embedded', use_embedded);
      mask Callback use_hdl:
      | use_hdl = get_param(gcb,'use_hdl');
      | if( strcmp(use_hdl,'on')),
      |     set_param(gcb, 'use_embedded','off');
      |     set_param(gcb, 'MaskVisibilities',{'on','on','on','on','off'});
      | else,
      |     set_param(gcb, 'MaskVisibilities',{'on','on','on','on','on'});
      | end
  pol1_in1_last_tap9 : Subsystem  AncestorBlock=casper_library_pfbs/last_tap_real  mask(last_tap_real){BitWidthIn=16, CoeffBitWidth=16, mult_latency=2, use_hdl=on, use_embedded=off}
      mask prompts: BitWidthIn "Input Bitwidth:"; CoeffBitWidth "Coeff Bitwidth:"; mult_latency "Mult Latency"; use_hdl "Use behavioral HDL for multlipliers"; use_embedded "Use embedded multipliers"
      mask init:
      | last_tap_real_init(gcb,...
      |     'BitWidthIn', BitWidthIn,...
      |     'CoeffBitWidth', CoeffBitWidth,...
      |     'mult_latency', mult_latency,...
      |     'use_hdl', use_hdl,...
      |     'use_embedded', use_embedded);
      mask Callback use_hdl:
      | use_hdl = get_param(gcb,'use_hdl');
      | if( strcmp(use_hdl,'on')),
      |     set_param(gcb, 'use_embedded','off');
      |     set_param(gcb, 'MaskVisibilities',{'on','on','on','on','off'});
      | else,
      |     set_param(gcb, 'MaskVisibilities',{'on','on','on','on','on'});
      | end
  pol1_in1_tap1 : Subsystem  AncestorBlock=casper_library_pfbs/tap_real  mask(pfb_tap_real){mult_latency=2, coeff_width=16, coeff_frac_width=15, delay=16, data_width=16, bram_latency=2, use_hdl=on, use_embedded=off}
      mask prompts: mult_latency "Multiplier Latency"; coeff_width "Coefficient Bit Width In"; coeff_frac_width "Coefficient Fractional Bits"; delay "Data/Sync Delay"; data_width "Data Bit Width In"; bram_latency "BRAM Latency"; use_hdl "Use behavioral HDL for multlipliers"; use_embedded "Use embedded multipliers"
      mask init: same as rfsoc4x2_ospfb_128/pfb_fir_real10/pol1_in1_tap1
  pol1_in1_tap10 : Subsystem  AncestorBlock=casper_library_pfbs/tap_real  mask(pfb_tap_real){mult_latency=2, coeff_width=16, coeff_frac_width=15, delay=16, data_width=16, bram_latency=2, use_hdl=on, use_embedded=off}
      mask prompts: mult_latency "Multiplier Latency"; coeff_width "Coefficient Bit Width In"; coeff_frac_width "Coefficient Fractional Bits"; delay "Data/Sync Delay"; data_width "Data Bit Width In"; bram_latency "BRAM Latency"; use_hdl "Use behavioral HDL for multlipliers"; use_embedded "Use embedded multipliers"
      mask init: same as rfsoc4x2_ospfb_128/pfb_fir_real10/pol1_in1_tap1
  pol1_in1_tap11 : Subsystem  AncestorBlock=casper_library_pfbs/tap_real  mask(pfb_tap_real){mult_latency=2, coeff_width=16, coeff_frac_width=15, delay=16, data_width=16, bram_latency=2, use_hdl=on, use_embedded=off}
      mask prompts: mult_latency "Multiplier Latency"; coeff_width "Coefficient Bit Width In"; coeff_frac_width "Coefficient Fractional Bits"; delay "Data/Sync Delay"; data_width "Data Bit Width In"; bram_latency "BRAM Latency"; use_hdl "Use behavioral HDL for multlipliers"; use_embedded "Use embedded multipliers"
      mask init: same as rfsoc4x2_ospfb_128/pfb_fir_real10/pol1_in1_tap1
  pol1_in1_tap12 : Subsystem  AncestorBlock=casper_library_pfbs/tap_real  mask(pfb_tap_real){mult_latency=2, coeff_width=16, coeff_frac_width=15, delay=16, data_width=16, bram_latency=2, use_hdl=on, use_embedded=off}
      mask prompts: mult_latency "Multiplier Latency"; coeff_width "Coefficient Bit Width In"; coeff_frac_width "Coefficient Fractional Bits"; delay "Data/Sync Delay"; data_width "Data Bit Width In"; bram_latency "BRAM Latency"; use_hdl "Use behavioral HDL for multlipliers"; use_embedded "Use embedded multipliers"
      mask init: same as rfsoc4x2_ospfb_128/pfb_fir_real10/pol1_in1_tap1
  pol1_in1_tap13 : Subsystem  AncestorBlock=casper_library_pfbs/tap_real  mask(pfb_tap_real){mult_latency=2, coeff_width=16, coeff_frac_width=15, delay=16, data_width=16, bram_latency=2, use_hdl=on, use_embedded=off}
      mask prompts: mult_latency "Multiplier Latency"; coeff_width "Coefficient Bit Width In"; coeff_frac_width "Coefficient Fractional Bits"; delay "Data/Sync Delay"; data_width "Data Bit Width In"; bram_latency "BRAM Latency"; use_hdl "Use behavioral HDL for multlipliers"; use_embedded "Use embedded multipliers"
      mask init: same as rfsoc4x2_ospfb_128/pfb_fir_real10/pol1_in1_tap1
  pol1_in1_tap14 : Subsystem  AncestorBlock=casper_library_pfbs/tap_real  mask(pfb_tap_real){mult_latency=2, coeff_width=16, coeff_frac_width=15, delay=16, data_width=16, bram_latency=2, use_hdl=on, use_embedded=off}
      mask prompts: mult_latency "Multiplier Latency"; coeff_width "Coefficient Bit Width In"; coeff_frac_width "Coefficient Fractional Bits"; delay "Data/Sync Delay"; data_width "Data Bit Width In"; bram_latency "BRAM Latency"; use_hdl "Use behavioral HDL for multlipliers"; use_embedded "Use embedded multipliers"
      mask init: same as rfsoc4x2_ospfb_128/pfb_fir_real10/pol1_in1_tap1
  pol1_in1_tap15 : Subsystem  AncestorBlock=casper_library_pfbs/tap_real  mask(pfb_tap_real){mult_latency=2, coeff_width=16, coeff_frac_width=15, delay=16, data_width=16, bram_latency=2, use_hdl=on, use_embedded=off}
      mask prompts: mult_latency "Multiplier Latency"; coeff_width "Coefficient Bit Width In"; coeff_frac_width "Coefficient Fractional Bits"; delay "Data/Sync Delay"; data_width "Data Bit Width In"; bram_latency "BRAM Latency"; use_hdl "Use behavioral HDL for multlipliers"; use_embedded "Use embedded multipliers"
      mask init: same as rfsoc4x2_ospfb_128/pfb_fir_real10/pol1_in1_tap1
  pol1_in1_tap16 : Subsystem  AncestorBlock=casper_library_pfbs/tap_real  mask(pfb_tap_real){mult_latency=2, coeff_width=16, coeff_frac_width=15, delay=16, data_width=16, bram_latency=2, use_hdl=on, use_embedded=off}
      mask prompts: mult_latency "Multiplier Latency"; coeff_width "Coefficient Bit Width In"; coeff_frac_width "Coefficient Fractional Bits"; delay "Data/Sync Delay"; data_width "Data Bit Width In"; bram_latency "BRAM Latency"; use_hdl "Use behavioral HDL for multlipliers"; use_embedded "Use embedded multipliers"
      mask init: same as rfsoc4x2_ospfb_128/pfb_fir_real10/pol1_in1_tap1
  pol1_in1_tap17 : Subsystem  AncestorBlock=casper_library_pfbs/tap_real  mask(pfb_tap_real){mult_latency=2, coeff_width=16, coeff_frac_width=15, delay=16, data_width=16, bram_latency=2, use_hdl=on, use_embedded=off}
      mask prompts: mult_latency "Multiplier Latency"; coeff_width "Coefficient Bit Width In"; coeff_frac_width "Coefficient Fractional Bits"; delay "Data/Sync Delay"; data_width "Data Bit Width In"; bram_latency "BRAM Latency"; use_hdl "Use behavioral HDL for multlipliers"; use_embedded "Use embedded multipliers"
      mask init: same as rfsoc4x2_ospfb_128/pfb_fir_real10/pol1_in1_tap1
  pol1_in1_tap18 : Subsystem  AncestorBlock=casper_library_pfbs/tap_real  mask(pfb_tap_real){mult_latency=2, coeff_width=16, coeff_frac_width=15, delay=16, data_width=16, bram_latency=2, use_hdl=on, use_embedded=off}
      mask prompts: mult_latency "Multiplier Latency"; coeff_width "Coefficient Bit Width In"; coeff_frac_width "Coefficient Fractional Bits"; delay "Data/Sync Delay"; data_width "Data Bit Width In"; bram_latency "BRAM Latency"; use_hdl "Use behavioral HDL for multlipliers"; use_embedded "Use embedded multipliers"
      mask init: same as rfsoc4x2_ospfb_128/pfb_fir_real10/pol1_in1_tap1
  pol1_in1_tap19 : Subsystem  AncestorBlock=casper_library_pfbs/tap_real  mask(pfb_tap_real){mult_latency=2, coeff_width=16, coeff_frac_width=15, delay=16, data_width=16, bram_latency=2, use_hdl=on, use_embedded=off}
      mask prompts: mult_latency "Multiplier Latency"; coeff_width "Coefficient Bit Width In"; coeff_frac_width "Coefficient Fractional Bits"; delay "Data/Sync Delay"; data_width "Data Bit Width In"; bram_latency "BRAM Latency"; use_hdl "Use behavioral HDL for multlipliers"; use_embedded "Use embedded multipliers"
      mask init: same as rfsoc4x2_ospfb_128/pfb_fir_real10/pol1_in1_tap1
  pol1_in1_tap2 : Subsystem  AncestorBlock=casper_library_pfbs/tap_real  mask(pfb_tap_real){mult_latency=2, coeff_width=16, coeff_frac_width=15, delay=16, data_width=16, bram_latency=2, use_hdl=on, use_embedded=off}
      mask prompts: mult_latency "Multiplier Latency"; coeff_width "Coefficient Bit Width In"; coeff_frac_width "Coefficient Fractional Bits"; delay "Data/Sync Delay"; data_width "Data Bit Width In"; bram_latency "BRAM Latency"; use_hdl "Use behavioral HDL for multlipliers"; use_embedded "Use embedded multipliers"
      mask init: same as rfsoc4x2_ospfb_128/pfb_fir_real10/pol1_in1_tap1
  pol1_in1_tap20 : Subsystem  AncestorBlock=casper_library_pfbs/tap_real  mask(pfb_tap_real){mult_latency=2, coeff_width=16, coeff_frac_width=15, delay=16, data_width=16, bram_latency=2, use_hdl=on, use_embedded=off}
      mask prompts: mult_latency "Multiplier Latency"; coeff_width "Coefficient Bit Width In"; coeff_frac_width "Coefficient Fractional Bits"; delay "Data/Sync Delay"; data_width "Data Bit Width In"; bram_latency "BRAM Latency"; use_hdl "Use behavioral HDL for multlipliers"; use_embedded "Use embedded multipliers"
      mask init: same as rfsoc4x2_ospfb_128/pfb_fir_real10/pol1_in1_tap1
  pol1_in1_tap21 : Subsystem  AncestorBlock=casper_library_pfbs/tap_real  mask(pfb_tap_real){mult_latency=2, coeff_width=16, coeff_frac_width=15, delay=16, data_width=16, bram_latency=2, use_hdl=on, use_embedded=off}
      mask prompts: mult_latency "Multiplier Latency"; coeff_width "Coefficient Bit Width In"; coeff_frac_width "Coefficient Fractional Bits"; delay "Data/Sync Delay"; data_width "Data Bit Width In"; bram_latency "BRAM Latency"; use_hdl "Use behavioral HDL for multlipliers"; use_embedded "Use embedded multipliers"
      mask init: same as rfsoc4x2_ospfb_128/pfb_fir_real10/pol1_in1_tap1
  pol1_in1_tap22 : Subsystem  AncestorBlock=casper_library_pfbs/tap_real  mask(pfb_tap_real){mult_latency=2, coeff_width=16, coeff_frac_width=15, delay=16, data_width=16, bram_latency=2, use_hdl=on, use_embedded=off}
      mask prompts: mult_latency "Multiplier Latency"; coeff_width "Coefficient Bit Width In"; coeff_frac_width "Coefficient Fractional Bits"; delay "Data/Sync Delay"; data_width "Data Bit Width In"; bram_latency "BRAM Latency"; use_hdl "Use behavioral HDL for multlipliers"; use_embedded "Use embedded multipliers"
      mask init: same as rfsoc4x2_ospfb_128/pfb_fir_real10/pol1_in1_tap1
  pol1_in1_tap23 : Subsystem  AncestorBlock=casper_library_pfbs/tap_real  mask(pfb_tap_real){mult_latency=2, coeff_width=16, coeff_frac_width=15, delay=16, data_width=16, bram_latency=2, use_hdl=on, use_embedded=off}
      mask prompts: mult_latency "Multiplier Latency"; coeff_width "Coefficient Bit Width In"; coeff_frac_width "Coefficient Fractional Bits"; delay "Data/Sync Delay"; data_width "Data Bit Width In"; bram_latency "BRAM Latency"; use_hdl "Use behavioral HDL for multlipliers"; use_embedded "Use embedded multipliers"
      mask init: same as rfsoc4x2_ospfb_128/pfb_fir_real10/pol1_in1_tap1
  pol1_in1_tap24 : Subsystem  AncestorBlock=casper_library_pfbs/tap_real  mask(pfb_tap_real){mult_latency=2, coeff_width=16, coeff_frac_width=15, delay=16, data_width=16, bram_latency=2, use_hdl=on, use_embedded=off}
      mask prompts: mult_latency "Multiplier Latency"; coeff_width "Coefficient Bit Width In"; coeff_frac_width "Coefficient Fractional Bits"; delay "Data/Sync Delay"; data_width "Data Bit Width In"; bram_latency "BRAM Latency"; use_hdl "Use behavioral HDL for multlipliers"; use_embedded "Use embedded multipliers"
      mask init: same as rfsoc4x2_ospfb_128/pfb_fir_real10/pol1_in1_tap1
  pol1_in1_tap25 : Subsystem  AncestorBlock=casper_library_pfbs/tap_real  mask(pfb_tap_real){mult_latency=2, coeff_width=16, coeff_frac_width=15, delay=16, data_width=16, bram_latency=2, use_hdl=on, use_embedded=off}
      mask prompts: mult_latency "Multiplier Latency"; coeff_width "Coefficient Bit Width In"; coeff_frac_width "Coefficient Fractional Bits"; delay "Data/Sync Delay"; data_width "Data Bit Width In"; bram_latency "BRAM Latency"; use_hdl "Use behavioral HDL for multlipliers"; use_embedded "Use embedded multipliers"
      mask init: same as rfsoc4x2_ospfb_128/pfb_fir_real10/pol1_in1_tap1
  pol1_in1_tap26 : Subsystem  AncestorBlock=casper_library_pfbs/tap_real  mask(pfb_tap_real){mult_latency=2, coeff_width=16, coeff_frac_width=15, delay=16, data_width=16, bram_latency=2, use_hdl=on, use_embedded=off}
      mask prompts: mult_latency "Multiplier Latency"; coeff_width "Coefficient Bit Width In"; coeff_frac_width "Coefficient Fractional Bits"; delay "Data/Sync Delay"; data_width "Data Bit Width In"; bram_latency "BRAM Latency"; use_hdl "Use behavioral HDL for multlipliers"; use_embedded "Use embedded multipliers"
      mask init: same as rfsoc4x2_ospfb_128/pfb_fir_real10/pol1_in1_tap1
  pol1_in1_tap27 : Subsystem  AncestorBlock=casper_library_pfbs/tap_real  mask(pfb_tap_real){mult_latency=2, coeff_width=16, coeff_frac_width=15, delay=16, data_width=16, bram_latency=2, use_hdl=on, use_embedded=off}
      mask prompts: mult_latency "Multiplier Latency"; coeff_width "Coefficient Bit Width In"; coeff_frac_width "Coefficient Fractional Bits"; delay "Data/Sync Delay"; data_width "Data Bit Width In"; bram_latency "BRAM Latency"; use_hdl "Use behavioral HDL for multlipliers"; use_embedded "Use embedded multipliers"
      mask init: same as rfsoc4x2_ospfb_128/pfb_fir_real10/pol1_in1_tap1
  pol1_in1_tap28 : Subsystem  AncestorBlock=casper_library_pfbs/tap_real  mask(pfb_tap_real){mult_latency=2, coeff_width=16, coeff_frac_width=15, delay=16, data_width=16, bram_latency=2, use_hdl=on, use_embedded=off}
      mask prompts: mult_latency "Multiplier Latency"; coeff_width "Coefficient Bit Width In"; coeff_frac_width "Coefficient Fractional Bits"; delay "Data/Sync Delay"; data_width "Data Bit Width In"; bram_latency "BRAM Latency"; use_hdl "Use behavioral HDL for multlipliers"; use_embedded "Use embedded multipliers"
      mask init: same as rfsoc4x2_ospfb_128/pfb_fir_real10/pol1_in1_tap1
  pol1_in1_tap29 : Subsystem  AncestorBlock=casper_library_pfbs/tap_real  mask(pfb_tap_real){mult_latency=2, coeff_width=16, coeff_frac_width=15, delay=16, data_width=16, bram_latency=2, use_hdl=on, use_embedded=off}
      mask prompts: mult_latency "Multiplier Latency"; coeff_width "Coefficient Bit Width In"; coeff_frac_width "Coefficient Fractional Bits"; delay "Data/Sync Delay"; data_width "Data Bit Width In"; bram_latency "BRAM Latency"; use_hdl "Use behavioral HDL for multlipliers"; use_embedded "Use embedded multipliers"
      mask init: same as rfsoc4x2_ospfb_128/pfb_fir_real10/pol1_in1_tap1
  pol1_in1_tap3 : Subsystem  AncestorBlock=casper_library_pfbs/tap_real  mask(pfb_tap_real){mult_latency=2, coeff_width=16, coeff_frac_width=15, delay=16, data_width=16, bram_latency=2, use_hdl=on, use_embedded=off}
      mask prompts: mult_latency "Multiplier Latency"; coeff_width "Coefficient Bit Width In"; coeff_frac_width "Coefficient Fractional Bits"; delay "Data/Sync Delay"; data_width "Data Bit Width In"; bram_latency "BRAM Latency"; use_hdl "Use behavioral HDL for multlipliers"; use_embedded "Use embedded multipliers"
      mask init: same as rfsoc4x2_ospfb_128/pfb_fir_real10/pol1_in1_tap1
  pol1_in1_tap30 : Subsystem  AncestorBlock=casper_library_pfbs/tap_real  mask(pfb_tap_real){mult_latency=2, coeff_width=16, coeff_frac_width=15, delay=16, data_width=16, bram_latency=2, use_hdl=on, use_embedded=off}
      mask prompts: mult_latency "Multiplier Latency"; coeff_width "Coefficient Bit Width In"; coeff_frac_width "Coefficient Fractional Bits"; delay "Data/Sync Delay"; data_width "Data Bit Width In"; bram_latency "BRAM Latency"; use_hdl "Use behavioral HDL for multlipliers"; use_embedded "Use embedded multipliers"
      mask init: same as rfsoc4x2_ospfb_128/pfb_fir_real10/pol1_in1_tap1
  pol1_in1_tap31 : Subsystem  AncestorBlock=casper_library_pfbs/tap_real  mask(pfb_tap_real){mult_latency=2, coeff_width=16, coeff_frac_width=15, delay=16, data_width=16, bram_latency=2, use_hdl=on, use_embedded=off}
      mask prompts: mult_latency "Multiplier Latency"; coeff_width "Coefficient Bit Width In"; coeff_frac_width "Coefficient Fractional Bits"; delay "Data/Sync Delay"; data_width "Data Bit Width In"; bram_latency "BRAM Latency"; use_hdl "Use behavioral HDL for multlipliers"; use_embedded "Use embedded multipliers"
      mask init: same as rfsoc4x2_ospfb_128/pfb_fir_real10/pol1_in1_tap1
  pol1_in1_tap32 : Subsystem  AncestorBlock=casper_library_pfbs/tap_real  mask(pfb_tap_real){mult_latency=2, coeff_width=16, coeff_frac_width=15, delay=16, data_width=16, bram_latency=2, use_hdl=on, use_embedded=off}
      mask prompts: mult_latency "Multiplier Latency"; coeff_width "Coefficient Bit Width In"; coeff_frac_width "Coefficient Fractional Bits"; delay "Data/Sync Delay"; data_width "Data Bit Width In"; bram_latency "BRAM Latency"; use_hdl "Use behavioral HDL for multlipliers"; use_embedded "Use embedded multipliers"
      mask init: same as rfsoc4x2_ospfb_128/pfb_fir_real10/pol1_in1_tap1
  pol1_in1_tap33 : Subsystem  AncestorBlock=casper_library_pfbs/tap_real  mask(pfb_tap_real){mult_latency=2, coeff_width=16, coeff_frac_width=15, delay=16, data_width=16, bram_latency=2, use_hdl=on, use_embedded=off}
      mask prompts: mult_latency "Multiplier Latency"; coeff_width "Coefficient Bit Width In"; coeff_frac_width "Coefficient Fractional Bits"; delay "Data/Sync Delay"; data_width "Data Bit Width In"; bram_latency "BRAM Latency"; use_hdl "Use behavioral HDL for multlipliers"; use_embedded "Use embedded multipliers"
      mask init: same as rfsoc4x2_ospfb_128/pfb_fir_real10/pol1_in1_tap1
  pol1_in1_tap34 : Subsystem  AncestorBlock=casper_library_pfbs/tap_real  mask(pfb_tap_real){mult_latency=2, coeff_width=16, coeff_frac_width=15, delay=16, data_width=16, bram_latency=2, use_hdl=on, use_embedded=off}
      mask prompts: mult_latency "Multiplier Latency"; coeff_width "Coefficient Bit Width In"; coeff_frac_width "Coefficient Fractional Bits"; delay "Data/Sync Delay"; data_width "Data Bit Width In"; bram_latency "BRAM Latency"; use_hdl "Use behavioral HDL for multlipliers"; use_embedded "Use embedded multipliers"
      mask init: same as rfsoc4x2_ospfb_128/pfb_fir_real10/pol1_in1_tap1
  pol1_in1_tap35 : Subsystem  AncestorBlock=casper_library_pfbs/tap_real  mask(pfb_tap_real){mult_latency=2, coeff_width=16, coeff_frac_width=15, delay=16, data_width=16, bram_latency=2, use_hdl=on, use_embedded=off}
      mask prompts: mult_latency "Multiplier Latency"; coeff_width "Coefficient Bit Width In"; coeff_frac_width "Coefficient Fractional Bits"; delay "Data/Sync Delay"; data_width "Data Bit Width In"; bram_latency "BRAM Latency"; use_hdl "Use behavioral HDL for multlipliers"; use_embedded "Use embedded multipliers"
      mask init: same as rfsoc4x2_ospfb_128/pfb_fir_real10/pol1_in1_tap1
  pol1_in1_tap36 : Subsystem  AncestorBlock=casper_library_pfbs/tap_real  mask(pfb_tap_real){mult_latency=2, coeff_width=16, coeff_frac_width=15, delay=16, data_width=16, bram_latency=2, use_hdl=on, use_embedded=off}
      mask prompts: mult_latency "Multiplier Latency"; coeff_width "Coefficient Bit Width In"; coeff_frac_width "Coefficient Fractional Bits"; delay "Data/Sync Delay"; data_width "Data Bit Width In"; bram_latency "BRAM Latency"; use_hdl "Use behavioral HDL for multlipliers"; use_embedded "Use embedded multipliers"
      mask init: same as rfsoc4x2_ospfb_128/pfb_fir_real10/pol1_in1_tap1
  pol1_in1_tap37 : Subsystem  AncestorBlock=casper_library_pfbs/tap_real  mask(pfb_tap_real){mult_latency=2, coeff_width=16, coeff_frac_width=15, delay=16, data_width=16, bram_latency=2, use_hdl=on, use_embedded=off}
      mask prompts: mult_latency "Multiplier Latency"; coeff_width "Coefficient Bit Width In"; coeff_frac_width "Coefficient Fractional Bits"; delay "Data/Sync Delay"; data_width "Data Bit Width In"; bram_latency "BRAM Latency"; use_hdl "Use behavioral HDL for multlipliers"; use_embedded "Use embedded multipliers"
      mask init: same as rfsoc4x2_ospfb_128/pfb_fir_real10/pol1_in1_tap1
  pol1_in1_tap38 : Subsystem  AncestorBlock=casper_library_pfbs/tap_real  mask(pfb_tap_real){mult_latency=2, coeff_width=16, coeff_frac_width=15, delay=16, data_width=16, bram_latency=2, use_hdl=on, use_embedded=off}
      mask prompts: mult_latency "Multiplier Latency"; coeff_width "Coefficient Bit Width In"; coeff_frac_width "Coefficient Fractional Bits"; delay "Data/Sync Delay"; data_width "Data Bit Width In"; bram_latency "BRAM Latency"; use_hdl "Use behavioral HDL for multlipliers"; use_embedded "Use embedded multipliers"
      mask init: same as rfsoc4x2_ospfb_128/pfb_fir_real10/pol1_in1_tap1
  pol1_in1_tap39 : Subsystem  AncestorBlock=casper_library_pfbs/tap_real  mask(pfb_tap_real){mult_latency=2, coeff_width=16, coeff_frac_width=15, delay=16, data_width=16, bram_latency=2, use_hdl=on, use_embedded=off}
      mask prompts: mult_latency "Multiplier Latency"; coeff_width "Coefficient Bit Width In"; coeff_frac_width "Coefficient Fractional Bits"; delay "Data/Sync Delay"; data_width "Data Bit Width In"; bram_latency "BRAM Latency"; use_hdl "Use behavioral HDL for multlipliers"; use_embedded "Use embedded multipliers"
      mask init: same as rfsoc4x2_ospfb_128/pfb_fir_real10/pol1_in1_tap1
  pol1_in1_tap4 : Subsystem  AncestorBlock=casper_library_pfbs/tap_real  mask(pfb_tap_real){mult_latency=2, coeff_width=16, coeff_frac_width=15, delay=16, data_width=16, bram_latency=2, use_hdl=on, use_embedded=off}
      mask prompts: mult_latency "Multiplier Latency"; coeff_width "Coefficient Bit Width In"; coeff_frac_width "Coefficient Fractional Bits"; delay "Data/Sync Delay"; data_width "Data Bit Width In"; bram_latency "BRAM Latency"; use_hdl "Use behavioral HDL for multlipliers"; use_embedded "Use embedded multipliers"
      mask init: same as rfsoc4x2_ospfb_128/pfb_fir_real10/pol1_in1_tap1
  pol1_in1_tap40 : Subsystem  AncestorBlock=casper_library_pfbs/tap_real  mask(pfb_tap_real){mult_latency=2, coeff_width=16, coeff_frac_width=15, delay=16, data_width=16, bram_latency=2, use_hdl=on, use_embedded=off}
      mask prompts: mult_latency "Multiplier Latency"; coeff_width "Coefficient Bit Width In"; coeff_frac_width "Coefficient Fractional Bits"; delay "Data/Sync Delay"; data_width "Data Bit Width In"; bram_latency "BRAM Latency"; use_hdl "Use behavioral HDL for multlipliers"; use_embedded "Use embedded multipliers"
      mask init: same as rfsoc4x2_ospfb_128/pfb_fir_real10/pol1_in1_tap1
  pol1_in1_tap41 : Subsystem  AncestorBlock=casper_library_pfbs/tap_real  mask(pfb_tap_real){mult_latency=2, coeff_width=16, coeff_frac_width=15, delay=16, data_width=16, bram_latency=2, use_hdl=on, use_embedded=off}
      mask prompts: mult_latency "Multiplier Latency"; coeff_width "Coefficient Bit Width In"; coeff_frac_width "Coefficient Fractional Bits"; delay "Data/Sync Delay"; data_width "Data Bit Width In"; bram_latency "BRAM Latency"; use_hdl "Use behavioral HDL for multlipliers"; use_embedded "Use embedded multipliers"
      mask init: same as rfsoc4x2_ospfb_128/pfb_fir_real10/pol1_in1_tap1
  pol1_in1_tap42 : Subsystem  AncestorBlock=casper_library_pfbs/tap_real  mask(pfb_tap_real){mult_latency=2, coeff_width=16, coeff_frac_width=15, delay=16, data_width=16, bram_latency=2, use_hdl=on, use_embedded=off}
      mask prompts: mult_latency "Multiplier Latency"; coeff_width "Coefficient Bit Width In"; coeff_frac_width "Coefficient Fractional Bits"; delay "Data/Sync Delay"; data_width "Data Bit Width In"; bram_latency "BRAM Latency"; use_hdl "Use behavioral HDL for multlipliers"; use_embedded "Use embedded multipliers"
      mask init: same as rfsoc4x2_ospfb_128/pfb_fir_real10/pol1_in1_tap1
  pol1_in1_tap43 : Subsystem  AncestorBlock=casper_library_pfbs/tap_real  mask(pfb_tap_real){mult_latency=2, coeff_width=16, coeff_frac_width=15, delay=16, data_width=16, bram_latency=2, use_hdl=on, use_embedded=off}
      mask prompts: mult_latency "Multiplier Latency"; coeff_width "Coefficient Bit Width In"; coeff_frac_width "Coefficient Fractional Bits"; delay "Data/Sync Delay"; data_width "Data Bit Width In"; bram_latency "BRAM Latency"; use_hdl "Use behavioral HDL for multlipliers"; use_embedded "Use embedded multipliers"
      mask init: same as rfsoc4x2_ospfb_128/pfb_fir_real10/pol1_in1_tap1
  pol1_in1_tap44 : Subsystem  AncestorBlock=casper_library_pfbs/tap_real  mask(pfb_tap_real){mult_latency=2, coeff_width=16, coeff_frac_width=15, delay=16, data_width=16, bram_latency=2, use_hdl=on, use_embedded=off}
      mask prompts: mult_latency "Multiplier Latency"; coeff_width "Coefficient Bit Width In"; coeff_frac_width "Coefficient Fractional Bits"; delay "Data/Sync Delay"; data_width "Data Bit Width In"; bram_latency "BRAM Latency"; use_hdl "Use behavioral HDL for multlipliers"; use_embedded "Use embedded multipliers"
      mask init: same as rfsoc4x2_ospfb_128/pfb_fir_real10/pol1_in1_tap1
  pol1_in1_tap45 : Subsystem  AncestorBlock=casper_library_pfbs/tap_real  mask(pfb_tap_real){mult_latency=2, coeff_width=16, coeff_frac_width=15, delay=16, data_width=16, bram_latency=2, use_hdl=on, use_embedded=off}
      mask prompts: mult_latency "Multiplier Latency"; coeff_width "Coefficient Bit Width In"; coeff_frac_width "Coefficient Fractional Bits"; delay "Data/Sync Delay"; data_width "Data Bit Width In"; bram_latency "BRAM Latency"; use_hdl "Use behavioral HDL for multlipliers"; use_embedded "Use embedded multipliers"
      mask init: same as rfsoc4x2_ospfb_128/pfb_fir_real10/pol1_in1_tap1
  pol1_in1_tap46 : Subsystem  AncestorBlock=casper_library_pfbs/tap_real  mask(pfb_tap_real){mult_latency=2, coeff_width=16, coeff_frac_width=15, delay=16, data_width=16, bram_latency=2, use_hdl=on, use_embedded=off}
      mask prompts: mult_latency "Multiplier Latency"; coeff_width "Coefficient Bit Width In"; coeff_frac_width "Coefficient Fractional Bits"; delay "Data/Sync Delay"; data_width "Data Bit Width In"; bram_latency "BRAM Latency"; use_hdl "Use behavioral HDL for multlipliers"; use_embedded "Use embedded multipliers"
      mask init: same as rfsoc4x2_ospfb_128/pfb_fir_real10/pol1_in1_tap1
  pol1_in1_tap47 : Subsystem  AncestorBlock=casper_library_pfbs/tap_real  mask(pfb_tap_real){mult_latency=2, coeff_width=16, coeff_frac_width=15, delay=16, data_width=16, bram_latency=2, use_hdl=on, use_embedded=off}
      mask prompts: mult_latency "Multiplier Latency"; coeff_width "Coefficient Bit Width In"; coeff_frac_width "Coefficient Fractional Bits"; delay "Data/Sync Delay"; data_width "Data Bit Width In"; bram_latency "BRAM Latency"; use_hdl "Use behavioral HDL for multlipliers"; use_embedded "Use embedded multipliers"
      mask init: same as rfsoc4x2_ospfb_128/pfb_fir_real10/pol1_in1_tap1
  pol1_in1_tap48 : Subsystem  AncestorBlock=casper_library_pfbs/tap_real  mask(pfb_tap_real){mult_latency=2, coeff_width=16, coeff_frac_width=15, delay=16, data_width=16, bram_latency=2, use_hdl=on, use_embedded=off}
      mask prompts: mult_latency "Multiplier Latency"; coeff_width "Coefficient Bit Width In"; coeff_frac_width "Coefficient Fractional Bits"; delay "Data/Sync Delay"; data_width "Data Bit Width In"; bram_latency "BRAM Latency"; use_hdl "Use behavioral HDL for multlipliers"; use_embedded "Use embedded multipliers"
      mask init: same as rfsoc4x2_ospfb_128/pfb_fir_real10/pol1_in1_tap1
  pol1_in1_tap49 : Subsystem  AncestorBlock=casper_library_pfbs/tap_real  mask(pfb_tap_real){mult_latency=2, coeff_width=16, coeff_frac_width=15, delay=16, data_width=16, bram_latency=2, use_hdl=on, use_embedded=off}
      mask prompts: mult_latency "Multiplier Latency"; coeff_width "Coefficient Bit Width In"; coeff_frac_width "Coefficient Fractional Bits"; delay "Data/Sync Delay"; data_width "Data Bit Width In"; bram_latency "BRAM Latency"; use_hdl "Use behavioral HDL for multlipliers"; use_embedded "Use embedded multipliers"
      mask init: same as rfsoc4x2_ospfb_128/pfb_fir_real10/pol1_in1_tap1
  pol1_in1_tap5 : Subsystem  AncestorBlock=casper_library_pfbs/tap_real  mask(pfb_tap_real){mult_latency=2, coeff_width=16, coeff_frac_width=15, delay=16, data_width=16, bram_latency=2, use_hdl=on, use_embedded=off}
      mask prompts: mult_latency "Multiplier Latency"; coeff_width "Coefficient Bit Width In"; coeff_frac_width "Coefficient Fractional Bits"; delay "Data/Sync Delay"; data_width "Data Bit Width In"; bram_latency "BRAM Latency"; use_hdl "Use behavioral HDL for multlipliers"; use_embedded "Use embedded multipliers"
      mask init: same as rfsoc4x2_ospfb_128/pfb_fir_real10/pol1_in1_tap1
  pol1_in1_tap50 : Subsystem  AncestorBlock=casper_library_pfbs/tap_real  mask(pfb_tap_real){mult_latency=2, coeff_width=16, coeff_frac_width=15, delay=16, data_width=16, bram_latency=2, use_hdl=on, use_embedded=off}
      mask prompts: mult_latency "Multiplier Latency"; coeff_width "Coefficient Bit Width In"; coeff_frac_width "Coefficient Fractional Bits"; delay "Data/Sync Delay"; data_width "Data Bit Width In"; bram_latency "BRAM Latency"; use_hdl "Use behavioral HDL for multlipliers"; use_embedded "Use embedded multipliers"
      mask init: same as rfsoc4x2_ospfb_128/pfb_fir_real10/pol1_in1_tap1
  pol1_in1_tap51 : Subsystem  AncestorBlock=casper_library_pfbs/tap_real  mask(pfb_tap_real){mult_latency=2, coeff_width=16, coeff_frac_width=15, delay=16, data_width=16, bram_latency=2, use_hdl=on, use_embedded=off}
      mask prompts: mult_latency "Multiplier Latency"; coeff_width "Coefficient Bit Width In"; coeff_frac_width "Coefficient Fractional Bits"; delay "Data/Sync Delay"; data_width "Data Bit Width In"; bram_latency "BRAM Latency"; use_hdl "Use behavioral HDL for multlipliers"; use_embedded "Use embedded multipliers"
      mask init: same as rfsoc4x2_ospfb_128/pfb_fir_real10/pol1_in1_tap1
  pol1_in1_tap52 : Subsystem  AncestorBlock=casper_library_pfbs/tap_real  mask(pfb_tap_real){mult_latency=2, coeff_width=16, coeff_frac_width=15, delay=16, data_width=16, bram_latency=2, use_hdl=on, use_embedded=off}
      mask prompts: mult_latency "Multiplier Latency"; coeff_width "Coefficient Bit Width In"; coeff_frac_width "Coefficient Fractional Bits"; delay "Data/Sync Delay"; data_width "Data Bit Width In"; bram_latency "BRAM Latency"; use_hdl "Use behavioral HDL for multlipliers"; use_embedded "Use embedded multipliers"
      mask init: same as rfsoc4x2_ospfb_128/pfb_fir_real10/pol1_in1_tap1
  pol1_in1_tap53 : Subsystem  AncestorBlock=casper_library_pfbs/tap_real  mask(pfb_tap_real){mult_latency=2, coeff_width=16, coeff_frac_width=15, delay=16, data_width=16, bram_latency=2, use_hdl=on, use_embedded=off}
      mask prompts: mult_latency "Multiplier Latency"; coeff_width "Coefficient Bit Width In"; coeff_frac_width "Coefficient Fractional Bits"; delay "Data/Sync Delay"; data_width "Data Bit Width In"; bram_latency "BRAM Latency"; use_hdl "Use behavioral HDL for multlipliers"; use_embedded "Use embedded multipliers"
      mask init: same as rfsoc4x2_ospfb_128/pfb_fir_real10/pol1_in1_tap1
  pol1_in1_tap54 : Subsystem  AncestorBlock=casper_library_pfbs/tap_real  mask(pfb_tap_real){mult_latency=2, coeff_width=16, coeff_frac_width=15, delay=16, data_width=16, bram_latency=2, use_hdl=on, use_embedded=off}
      mask prompts: mult_latency "Multiplier Latency"; coeff_width "Coefficient Bit Width In"; coeff_frac_width "Coefficient Fractional Bits"; delay "Data/Sync Delay"; data_width "Data Bit Width In"; bram_latency "BRAM Latency"; use_hdl "Use behavioral HDL for multlipliers"; use_embedded "Use embedded multipliers"
      mask init: same as rfsoc4x2_ospfb_128/pfb_fir_real10/pol1_in1_tap1
  pol1_in1_tap55 : Subsystem  AncestorBlock=casper_library_pfbs/tap_real  mask(pfb_tap_real){mult_latency=2, coeff_width=16, coeff_frac_width=15, delay=16, data_width=16, bram_latency=2, use_hdl=on, use_embedded=off}
      mask prompts: mult_latency "Multiplier Latency"; coeff_width "Coefficient Bit Width In"; coeff_frac_width "Coefficient Fractional Bits"; delay "Data/Sync Delay"; data_width "Data Bit Width In"; bram_latency "BRAM Latency"; use_hdl "Use behavioral HDL for multlipliers"; use_embedded "Use embedded multipliers"
      mask init: same as rfsoc4x2_ospfb_128/pfb_fir_real10/pol1_in1_tap1
  pol1_in1_tap56 : Subsystem  AncestorBlock=casper_library_pfbs/tap_real  mask(pfb_tap_real){mult_latency=2, coeff_width=16, coeff_frac_width=15, delay=16, data_width=16, bram_latency=2, use_hdl=on, use_embedded=off}
      mask prompts: mult_latency "Multiplier Latency"; coeff_width "Coefficient Bit Width In"; coeff_frac_width "Coefficient Fractional Bits"; delay "Data/Sync Delay"; data_width "Data Bit Width In"; bram_latency "BRAM Latency"; use_hdl "Use behavioral HDL for multlipliers"; use_embedded "Use embedded multipliers"
      mask init: same as rfsoc4x2_ospfb_128/pfb_fir_real10/pol1_in1_tap1
  pol1_in1_tap57 : Subsystem  AncestorBlock=casper_library_pfbs/tap_real  mask(pfb_tap_real){mult_latency=2, coeff_width=16, coeff_frac_width=15, delay=16, data_width=16, bram_latency=2, use_hdl=on, use_embedded=off}
      mask prompts: mult_latency "Multiplier Latency"; coeff_width "Coefficient Bit Width In"; coeff_frac_width "Coefficient Fractional Bits"; delay "Data/Sync Delay"; data_width "Data Bit Width In"; bram_latency "BRAM Latency"; use_hdl "Use behavioral HDL for multlipliers"; use_embedded "Use embedded multipliers"
      mask init: same as rfsoc4x2_ospfb_128/pfb_fir_real10/pol1_in1_tap1
  pol1_in1_tap58 : Subsystem  AncestorBlock=casper_library_pfbs/tap_real  mask(pfb_tap_real){mult_latency=2, coeff_width=16, coeff_frac_width=15, delay=16, data_width=16, bram_latency=2, use_hdl=on, use_embedded=off}
      mask prompts: mult_latency "Multiplier Latency"; coeff_width "Coefficient Bit Width In"; coeff_frac_width "Coefficient Fractional Bits"; delay "Data/Sync Delay"; data_width "Data Bit Width In"; bram_latency "BRAM Latency"; use_hdl "Use behavioral HDL for multlipliers"; use_embedded "Use embedded multipliers"
      mask init: same as rfsoc4x2_ospfb_128/pfb_fir_real10/pol1_in1_tap1
  pol1_in1_tap59 : Subsystem  AncestorBlock=casper_library_pfbs/tap_real  mask(pfb_tap_real){mult_latency=2, coeff_width=16, coeff_frac_width=15, delay=16, data_width=16, bram_latency=2, use_hdl=on, use_embedded=off}
      mask prompts: mult_latency "Multiplier Latency"; coeff_width "Coefficient Bit Width In"; coeff_frac_width "Coefficient Fractional Bits"; delay "Data/Sync Delay"; data_width "Data Bit Width In"; bram_latency "BRAM Latency"; use_hdl "Use behavioral HDL for multlipliers"; use_embedded "Use embedded multipliers"
      mask init: same as rfsoc4x2_ospfb_128/pfb_fir_real10/pol1_in1_tap1
  pol1_in1_tap6 : Subsystem  AncestorBlock=casper_library_pfbs/tap_real  mask(pfb_tap_real){mult_latency=2, coeff_width=16, coeff_frac_width=15, delay=16, data_width=16, bram_latency=2, use_hdl=on, use_embedded=off}
      mask prompts: mult_latency "Multiplier Latency"; coeff_width "Coefficient Bit Width In"; coeff_frac_width "Coefficient Fractional Bits"; delay "Data/Sync Delay"; data_width "Data Bit Width In"; bram_latency "BRAM Latency"; use_hdl "Use behavioral HDL for multlipliers"; use_embedded "Use embedded multipliers"
      mask init: same as rfsoc4x2_ospfb_128/pfb_fir_real10/pol1_in1_tap1
  pol1_in1_tap60 : Subsystem  AncestorBlock=casper_library_pfbs/tap_real  mask(pfb_tap_real){mult_latency=2, coeff_width=16, coeff_frac_width=15, delay=16, data_width=16, bram_latency=2, use_hdl=on, use_embedded=off}
      mask prompts: mult_latency "Multiplier Latency"; coeff_width "Coefficient Bit Width In"; coeff_frac_width "Coefficient Fractional Bits"; delay "Data/Sync Delay"; data_width "Data Bit Width In"; bram_latency "BRAM Latency"; use_hdl "Use behavioral HDL for multlipliers"; use_embedded "Use embedded multipliers"
      mask init: same as rfsoc4x2_ospfb_128/pfb_fir_real10/pol1_in1_tap1
  pol1_in1_tap61 : Subsystem  AncestorBlock=casper_library_pfbs/tap_real  mask(pfb_tap_real){mult_latency=2, coeff_width=16, coeff_frac_width=15, delay=16, data_width=16, bram_latency=2, use_hdl=on, use_embedded=off}
      mask prompts: mult_latency "Multiplier Latency"; coeff_width "Coefficient Bit Width In"; coeff_frac_width "Coefficient Fractional Bits"; delay "Data/Sync Delay"; data_width "Data Bit Width In"; bram_latency "BRAM Latency"; use_hdl "Use behavioral HDL for multlipliers"; use_embedded "Use embedded multipliers"
      mask init: same as rfsoc4x2_ospfb_128/pfb_fir_real10/pol1_in1_tap1
  pol1_in1_tap62 : Subsystem  AncestorBlock=casper_library_pfbs/tap_real  mask(pfb_tap_real){mult_latency=2, coeff_width=16, coeff_frac_width=15, delay=16, data_width=16, bram_latency=2, use_hdl=on, use_embedded=off}
      mask prompts: mult_latency "Multiplier Latency"; coeff_width "Coefficient Bit Width In"; coeff_frac_width "Coefficient Fractional Bits"; delay "Data/Sync Delay"; data_width "Data Bit Width In"; bram_latency "BRAM Latency"; use_hdl "Use behavioral HDL for multlipliers"; use_embedded "Use embedded multipliers"
      mask init: same as rfsoc4x2_ospfb_128/pfb_fir_real10/pol1_in1_tap1
  pol1_in1_tap63 : Subsystem  AncestorBlock=casper_library_pfbs/tap_real  mask(pfb_tap_real){mult_latency=2, coeff_width=16, coeff_frac_width=15, delay=16, data_width=16, bram_latency=2, use_hdl=on, use_embedded=off}
      mask prompts: mult_latency "Multiplier Latency"; coeff_width "Coefficient Bit Width In"; coeff_frac_width "Coefficient Fractional Bits"; delay "Data/Sync Delay"; data_width "Data Bit Width In"; bram_latency "BRAM Latency"; use_hdl "Use behavioral HDL for multlipliers"; use_embedded "Use embedded multipliers"
      mask init: same as rfsoc4x2_ospfb_128/pfb_fir_real10/pol1_in1_tap1
  pol1_in1_tap64 : Subsystem  AncestorBlock=casper_library_pfbs/tap_real  mask(pfb_tap_real){mult_latency=2, coeff_width=16, coeff_frac_width=15, delay=16, data_width=16, bram_latency=2, use_hdl=on, use_embedded=off}
      mask prompts: mult_latency "Multiplier Latency"; coeff_width "Coefficient Bit Width In"; coeff_frac_width "Coefficient Fractional Bits"; delay "Data/Sync Delay"; data_width "Data Bit Width In"; bram_latency "BRAM Latency"; use_hdl "Use behavioral HDL for multlipliers"; use_embedded "Use embedded multipliers"
      mask init: same as rfsoc4x2_ospfb_128/pfb_fir_real10/pol1_in1_tap1
  pol1_in1_tap65 : Subsystem  AncestorBlock=casper_library_pfbs/tap_real  mask(pfb_tap_real){mult_latency=2, coeff_width=16, coeff_frac_width=15, delay=16, data_width=16, bram_latency=2, use_hdl=on, use_embedded=off}
      mask prompts: mult_latency "Multiplier Latency"; coeff_width "Coefficient Bit Width In"; coeff_frac_width "Coefficient Fractional Bits"; delay "Data/Sync Delay"; data_width "Data Bit Width In"; bram_latency "BRAM Latency"; use_hdl "Use behavioral HDL for multlipliers"; use_embedded "Use embedded multipliers"
      mask init: same as rfsoc4x2_ospfb_128/pfb_fir_real10/pol1_in1_tap1
  pol1_in1_tap66 : Subsystem  AncestorBlock=casper_library_pfbs/tap_real  mask(pfb_tap_real){mult_latency=2, coeff_width=16, coeff_frac_width=15, delay=16, data_width=16, bram_latency=2, use_hdl=on, use_embedded=off}
      mask prompts: mult_latency "Multiplier Latency"; coeff_width "Coefficient Bit Width In"; coeff_frac_width "Coefficient Fractional Bits"; delay "Data/Sync Delay"; data_width "Data Bit Width In"; bram_latency "BRAM Latency"; use_hdl "Use behavioral HDL for multlipliers"; use_embedded "Use embedded multipliers"
      mask init: same as rfsoc4x2_ospfb_128/pfb_fir_real10/pol1_in1_tap1
  pol1_in1_tap67 : Subsystem  AncestorBlock=casper_library_pfbs/tap_real  mask(pfb_tap_real){mult_latency=2, coeff_width=16, coeff_frac_width=15, delay=16, data_width=16, bram_latency=2, use_hdl=on, use_embedded=off}
      mask prompts: mult_latency "Multiplier Latency"; coeff_width "Coefficient Bit Width In"; coeff_frac_width "Coefficient Fractional Bits"; delay "Data/Sync Delay"; data_width "Data Bit Width In"; bram_latency "BRAM Latency"; use_hdl "Use behavioral HDL for multlipliers"; use_embedded "Use embedded multipliers"
      mask init: same as rfsoc4x2_ospfb_128/pfb_fir_real10/pol1_in1_tap1
  pol1_in1_tap68 : Subsystem  AncestorBlock=casper_library_pfbs/tap_real  mask(pfb_tap_real){mult_latency=2, coeff_width=16, coeff_frac_width=15, delay=16, data_width=16, bram_latency=2, use_hdl=on, use_embedded=off}
      mask prompts: mult_latency "Multiplier Latency"; coeff_width "Coefficient Bit Width In"; coeff_frac_width "Coefficient Fractional Bits"; delay "Data/Sync Delay"; data_width "Data Bit Width In"; bram_latency "BRAM Latency"; use_hdl "Use behavioral HDL for multlipliers"; use_embedded "Use embedded multipliers"
      mask init: same as rfsoc4x2_ospfb_128/pfb_fir_real10/pol1_in1_tap1
  pol1_in1_tap69 : Subsystem  AncestorBlock=casper_library_pfbs/tap_real  mask(pfb_tap_real){mult_latency=2, coeff_width=16, coeff_frac_width=15, delay=16, data_width=16, bram_latency=2, use_hdl=on, use_embedded=off}
      mask prompts: mult_latency "Multiplier Latency"; coeff_width "Coefficient Bit Width In"; coeff_frac_width "Coefficient Fractional Bits"; delay "Data/Sync Delay"; data_width "Data Bit Width In"; bram_latency "BRAM Latency"; use_hdl "Use behavioral HDL for multlipliers"; use_embedded "Use embedded multipliers"
      mask init: same as rfsoc4x2_ospfb_128/pfb_fir_real10/pol1_in1_tap1
  pol1_in1_tap7 : Subsystem  AncestorBlock=casper_library_pfbs/tap_real  mask(pfb_tap_real){mult_latency=2, coeff_width=16, coeff_frac_width=15, delay=16, data_width=16, bram_latency=2, use_hdl=on, use_embedded=off}
      mask prompts: mult_latency "Multiplier Latency"; coeff_width "Coefficient Bit Width In"; coeff_frac_width "Coefficient Fractional Bits"; delay "Data/Sync Delay"; data_width "Data Bit Width In"; bram_latency "BRAM Latency"; use_hdl "Use behavioral HDL for multlipliers"; use_embedded "Use embedded multipliers"
      mask init: same as rfsoc4x2_ospfb_128/pfb_fir_real10/pol1_in1_tap1
  pol1_in1_tap70 : Subsystem  AncestorBlock=casper_library_pfbs/tap_real  mask(pfb_tap_real){mult_latency=2, coeff_width=16, coeff_frac_width=15, delay=16, data_width=16, bram_latency=2, use_hdl=on, use_embedded=off}
      mask prompts: mult_latency "Multiplier Latency"; coeff_width "Coefficient Bit Width In"; coeff_frac_width "Coefficient Fractional Bits"; delay "Data/Sync Delay"; data_width "Data Bit Width In"; bram_latency "BRAM Latency"; use_hdl "Use behavioral HDL for multlipliers"; use_embedded "Use embedded multipliers"
      mask init: same as rfsoc4x2_ospfb_128/pfb_fir_real10/pol1_in1_tap1
  pol1_in1_tap71 : Subsystem  AncestorBlock=casper_library_pfbs/tap_real  mask(pfb_tap_real){mult_latency=2, coeff_width=16, coeff_frac_width=15, delay=16, data_width=16, bram_latency=2, use_hdl=on, use_embedded=off}
      mask prompts: mult_latency "Multiplier Latency"; coeff_width "Coefficient Bit Width In"; coeff_frac_width "Coefficient Fractional Bits"; delay "Data/Sync Delay"; data_width "Data Bit Width In"; bram_latency "BRAM Latency"; use_hdl "Use behavioral HDL for multlipliers"; use_embedded "Use embedded multipliers"
      mask init: same as rfsoc4x2_ospfb_128/pfb_fir_real10/pol1_in1_tap1
  pol1_in1_tap72 : Subsystem  AncestorBlock=casper_library_pfbs/tap_real  mask(pfb_tap_real){mult_latency=2, coeff_width=16, coeff_frac_width=15, delay=16, data_width=16, bram_latency=2, use_hdl=on, use_embedded=off}
      mask prompts: mult_latency "Multiplier Latency"; coeff_width "Coefficient Bit Width In"; coeff_frac_width "Coefficient Fractional Bits"; delay "Data/Sync Delay"; data_width "Data Bit Width In"; bram_latency "BRAM Latency"; use_hdl "Use behavioral HDL for multlipliers"; use_embedded "Use embedded multipliers"
      mask init: same as rfsoc4x2_ospfb_128/pfb_fir_real10/pol1_in1_tap1
  pol1_in1_tap73 : Subsystem  AncestorBlock=casper_library_pfbs/tap_real  mask(pfb_tap_real){mult_latency=2, coeff_width=16, coeff_frac_width=15, delay=16, data_width=16, bram_latency=2, use_hdl=on, use_embedded=off}
      mask prompts: mult_latency "Multiplier Latency"; coeff_width "Coefficient Bit Width In"; coeff_frac_width "Coefficient Fractional Bits"; delay "Data/Sync Delay"; data_width "Data Bit Width In"; bram_latency "BRAM Latency"; use_hdl "Use behavioral HDL for multlipliers"; use_embedded "Use embedded multipliers"
      mask init: same as rfsoc4x2_ospfb_128/pfb_fir_real10/pol1_in1_tap1
  pol1_in1_tap74 : Subsystem  AncestorBlock=casper_library_pfbs/tap_real  mask(pfb_tap_real){mult_latency=2, coeff_width=16, coeff_frac_width=15, delay=16, data_width=16, bram_latency=2, use_hdl=on, use_embedded=off}
      mask prompts: mult_latency "Multiplier Latency"; coeff_width "Coefficient Bit Width In"; coeff_frac_width "Coefficient Fractional Bits"; delay "Data/Sync Delay"; data_width "Data Bit Width In"; bram_latency "BRAM Latency"; use_hdl "Use behavioral HDL for multlipliers"; use_embedded "Use embedded multipliers"
      mask init: same as rfsoc4x2_ospfb_128/pfb_fir_real10/pol1_in1_tap1
  pol1_in1_tap75 : Subsystem  AncestorBlock=casper_library_pfbs/tap_real  mask(pfb_tap_real){mult_latency=2, coeff_width=16, coeff_frac_width=15, delay=16, data_width=16, bram_latency=2, use_hdl=on, use_embedded=off}
      mask prompts: mult_latency "Multiplier Latency"; coeff_width "Coefficient Bit Width In"; coeff_frac_width "Coefficient Fractional Bits"; delay "Data/Sync Delay"; data_width "Data Bit Width In"; bram_latency "BRAM Latency"; use_hdl "Use behavioral HDL for multlipliers"; use_embedded "Use embedded multipliers"
      mask init: same as rfsoc4x2_ospfb_128/pfb_fir_real10/pol1_in1_tap1
  pol1_in1_tap76 : Subsystem  AncestorBlock=casper_library_pfbs/tap_real  mask(pfb_tap_real){mult_latency=2, coeff_width=16, coeff_frac_width=15, delay=16, data_width=16, bram_latency=2, use_hdl=on, use_embedded=off}
